simulink model "MMC_30_VSG_AD"  (R2023b)
settings: Solver=ode23t  StartTime=0.0  StopTime=2.4  RelTol=1e-3
InitFcn:
  | Rf=0.5929;
  | fn=50;
  | w0=2*pi*fn;
  | Lf=0.5*0.0135+0.01358;
  | R=0.5;
  | kf=8.5;
  | 
  | Kd=1.40543e+07;
  | lam=10; z0=0.707; zmax=1; wn0=lam/z0;
  | J0=223.613; DS0=4472.27;
  | Jmin=0.3*J0; Jmax=2.0*J0; Dmin=0.3*DS0; Dmax=2.2*DS0;
  | muJ=2906.97;
  | nu=0.15; nb=0.55; dzr=0.5; dzd=0;
  | tau=0.02; db=0.02; kpsi=14; txi=0.04;
  | Ts=0.0002; qref=0.03; dfref=0.064; dwref=0.4; dref=4;
  | lam_floor=1; scheme=1;
  | delta0=0.0712129;
  | J=J0; D=DS0;
libraries: spsIGBTDiodeLib x264, spsSeriesRLCBranchLib x140, spsVoltageMeasurementLib x132, spsCurrentMeasurementLib x6, spsSecondOrderFilterLib x3, spsThreePhaseVIMeasurementLib x2, spsDCVoltageSourceLib x2, slpidlib x2, spsGroundLib x1, spsPower3phInstantaneousLib x1, spsThreePhaseProgrammableVoltageSourceLib x1, spsThreePhaseSeriesRLCBranchLib x1
(part 1 of 5)
settings Model: Creator=LENOVO  LastModifiedBy=Lenovo
settings DataIOCC: ReturnWorkspaceOutputs=off

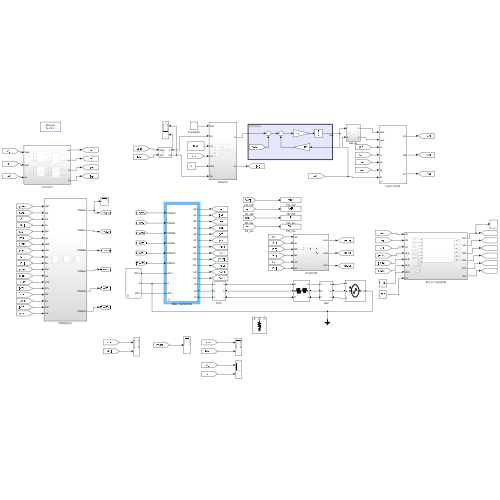
[thumbnail: Simulink's stored preview of the top-level diagram]
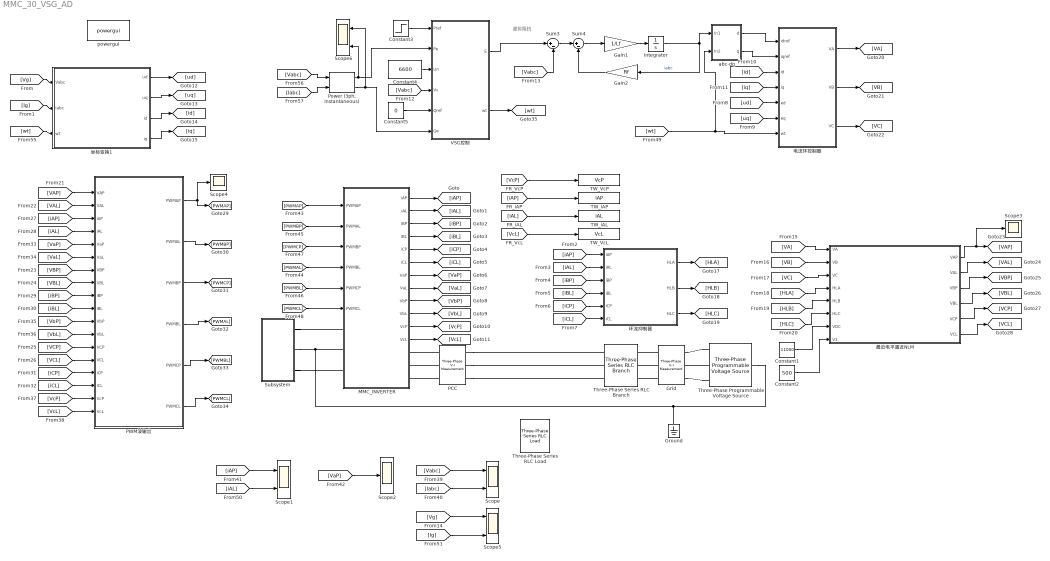
== system MMC_30_VSG_AD ==
  note: 虚拟阻抗
  Constant1 : Constant  Value=11000
  Constant2 : Constant  Value=500
  Constant3 : Step  Time=1.3  Before=1e6  After=1.1e6  SampleTime=0
  Constant4 : Constant  Value=6600
  Constant5 : Constant  Value=0
  Gain1 : Gain  Gain=1/Lf
  Gain2 : Gain  Gain=Rf
  Grid : spsThreePhaseVIMeasurementLib/Three-Phase V-I Measurement  VoltageMeasurement=phase-to-ground  SetLabelV=on  LabelV=Vg  Vpu=off  VpuLL=off  CurrentMeasurement=yes  SetLabelI=on  LabelI=Ig  Ipu=off  Pbase=100e6  Vbase=500e3  OutputType=Complex  PhasorSimulation=off  PSBequivalent=0
  Ground : spsGroundLib/Ground  LConnTagsString=a
  Integrator : Integrator
  MMC_INVERTER : Subsystem  mask{C0=4.7e-3, V0=500, L0=0.0135, C1=1e-3, R1=1e-6, V1=3500}
      mask prompts: C0 "旁路电容C0："; V0 "子模块初始电压V0："; L0 "桥臂电感L0："; C1 "直流电容C1："; R1 "电阻R1："; V1 "直流电容初始电压V1："
      mask DialogControl ParameterGroupVar Prompt: 参数
  PCC : spsThreePhaseVIMeasurementLib/Three-Phase V-I Measurement  VoltageMeasurement=phase-to-ground  SetLabelV=on  LabelV=Vabc  Vpu=off  VpuLL=off  CurrentMeasurement=yes  SetLabelI=on  LabelI=Iabc  Ipu=off  Pbase=100e6  Vbase=500e3  OutputType=Complex  PhasorSimulation=off  PSBequivalent=0
  PWM波输出 : Subsystem
  "Power (3ph, Instantaneous)" : spsPower3phInstantaneousLib/Power (3ph, Instantaneous)
  Scope{,1,5..6} (4 alike) : Scope  NumInputPorts=2
  Scope2 : Scope
  Scope3 : Scope
  Scope4 : Scope
  Subsystem : Subsystem  mask{VDC=11000}
      mask prompts: VDC "直流电压VDC："
      mask DialogControl ParameterGroupVar Prompt: 参数
  Sum3 : Sum  Inputs=|+-
  Sum4 : Sum  Inputs=|+-
  TW_VcL : ToWorkspace  VariableName=VcL  SaveFormat=Timeseries  SampleTime=Ts
  TW_VcP : ToWorkspace  VariableName=VcP  SaveFormat=Timeseries  SampleTime=Ts
  TW_iAL : ToWorkspace  VariableName=iAL  SaveFormat=Timeseries  SampleTime=Ts
  TW_iAP : ToWorkspace  VariableName=iAP  SaveFormat=Timeseries  SampleTime=Ts
  Three-Phase Programmable Voltage Source : spsThreePhaseProgrammableVoltageSourceLib/Three-Phase Programmable Voltage Source  PositiveSequence="[6600  0 50]"  VariationEntity=None  VariationType=Step  VariationTypeAlt=Step  VariationStep=-0.02  VariationRate=10  VariationMagnitude=0.3  VariationFrequency=2  VariationTiming=[1 2]  VariationPhaseA=off  Amplitudes=[1 0.8 1.2 1.0]  TimeValues=[0 0.1 0.15 0.2]  HarmonicGeneration=off  HarmonicA=[3 0.2 -25 0]  HarmonicB=[2 0.15 35 2]  Timing="[0.05  3]"  BusType=swing  Pref=0  Qref=0  Qmin=-inf  Qmax=inf
  Three-Phase Series RLC Branch : spsThreePhaseSeriesRLCBranchLib/Three-Phase Series RLC Branch  LConnTagsString=A|B|C  RConnTagsString=A|B|C  BranchType=RL  Resistance=0.5929  Inductance=13.58e-3  Capacitance=1e-6  Measurements=None
  Three-Phase Series RLC Load : spsThreePhaseSeriesRLCLoadLib/Three-Phase Series RLC Load  LConnTagsString=A|B|C  Configuration=Y (grounded)  NominalVoltage=6600  Vabc=[1e3 1e3 1e3]  Vabcp=[1e3 1e3 1e3]  NominalFrequency=50  UnbalancedPower=off  ActivePower=200e3  InductivePower=0  CapacitivePower=0  Pabc=[10e3 9e3 11e3]  QLabc=[100 90 110]  QCabc=[100 90 110]  Pabcp=[10e3 9e3 11e3]  QLabcp=[100 90 110]  QCabcp=[100 90 110]  Measurements=None  LoadType=constant Z
  VSG控制 : Subsystem
  abc-dq : Subsystem
  powergui : spspowerguiLib/powergui  Priority=1  SimulationMode=Discrete  SampleTime=5e-5  frequency=60  Iterations=50  frequencyindice=0  Pbase=100e6  ErrMax=1e-4  UnitsV=kV  UnitsW=MW  buscounter=0  FunctionMessages=off  echomessages=off  EnableUseOfTLC=off  CurrentSourceSwitches=off  DisableSnubberDevices=off  DisableRonSwitches=off  DisableVfSwitches=off  DisplayEquations=off  AutomaticDiscreteSolvers=off  SolverType=Tustin/Backward Euler (TBE)  Interpol=off  ExternalGateDelay=off  methode=off  Ts=100  x0status=blocks  SPID=on  SwTol=0  HookPort=off  NonlinearTolerance=1e-4  nMaxIteration=100  ContinueOnMaxIteration=off  RestoreLinks=warning  ResistiveCurrentMeasurement=off  Frange=[0:2:500]  Ylog=off  Xlog=on  ShowGrid=off  save=off  variable=ZData  structure=0  ZoomFFT=off  StartTime=0.0  cycles=1  DisplayStyle=1  fundamental=60  FreqAxis=off  MaxFrequency=1000  frequencyindicesteady=1  RmsSteady=1  display=off
  坐标变换1 : Subsystem
  最近电平逼近NLM : Subsystem
  环流抑制器 : Subsystem
  电流环控制器 : Subsystem  mask{Kp2=13.857, Ki2=58.576, wL=(0.0135/2+0.01358)*100*pi}
      mask prompts: Kp2 "电流内环Kp2："; Ki2 "电流内环Ki2："; wL "耦合量wL："
      mask DialogControl ParameterGroupVar Prompt: 参数
  wires:
  MMC_INVERTER/1(iAP) -> [iAP]
  MMC_INVERTER/2(iAL) -> [iAL]
  MMC_INVERTER/3(iBP) -> [iBP]
  MMC_INVERTER/4(iBL) -> [iBL]
  MMC_INVERTER/5(iCP) -> [iCP]
  MMC_INVERTER/6(iCL) -> [iCL]
  MMC_INVERTER/7(VaP) -> [VaP]
  MMC_INVERTER/12(VcL) -> [VcL]
  MMC_INVERTER/11(VcP) -> [VcP]
  MMC_INVERTER/10(VbL) -> [VbL]
  MMC_INVERTER/9(VbP) -> [VbP]
  MMC_INVERTER/8(VaL) -> [VaL]
  [Vg] -> 坐标变换1/1(Vabc)
  [Ig] -> 坐标变换1/2(Iabc)
  坐标变换1/1(ud) -> [ud]
  坐标变换1/2(uq) -> [uq]
  坐标变换1/3(id) -> [id]
  坐标变换1/4(iq) -> [iq]
  [iAP] -> 环流抑制器/1(iAP)
  [iAL] -> 环流抑制器/2(iAL)
  [iBP] -> 环流抑制器/3(iBP)
  [iBL] -> 环流抑制器/4(iBL)
  [iCP] -> 环流抑制器/5(iCP)
  [iCL] -> 环流抑制器/6(iCL)
  环流抑制器/1(HLA) -> [HLA]
  环流抑制器/2(HLB) -> [HLB]
  环流抑制器/3(HLC) -> [HLC]
  [id] -> 电流环控制器/3(id)
  [iq] -> 电流环控制器/4(iq)
  [ud] -> 电流环控制器/5(ed)
  [uq] -> 电流环控制器/6(eq)
  电流环控制器/1(VA) -> [VA]
  电流环控制器/2(VB) -> [VB]
  电流环控制器/3(VC) -> [VC]
  [VAP] -> PWM波输出/1(VAP)
  [VAL] -> PWM波输出/2(VAL)
  [VBP] -> PWM波输出/7(VBP)
  [VBL] -> PWM波输出/8(VBL)
  [VCP] -> PWM波输出/13(VCP)
  [VCL] -> PWM波输出/14(VCL)
  [iAP] -> PWM波输出/3(iAP)
  [iAL] -> PWM波输出/4(iAL)
  [VaP] -> PWM波输出/5(VaP)
  [VaL] -> PWM波输出/6(VaL)
  [iBP] -> PWM波输出/9(iBP)
  [iBL] -> PWM波输出/10(iBL)
  [VbP] -> PWM波输出/11(VbP)
  [VbL] -> PWM波输出/12(VbL)
  [iCP] -> PWM波输出/15(iCP)
  [iCL] -> PWM波输出/16(iCL)
  [VcP] -> PWM波输出/17(VcP)
  [VcL] -> PWM波输出/18(VcL)
  [Vabc] -> Scope/1
  [Iabc] -> Scope/2
  [iAP] -> Scope1/1
  [VaP] -> Scope2/1
  PWM波输出/6(PWMCL) -> [PWMCL]
  PWM波输出/4(PWMBL) -> [PWMAL]
  PWM波输出/5(PWMCP) -> [PWMBL]
  PWM波输出/1(PWMAP) -> [PWMAP], Scope4/1
  PWM波输出/3(PWMBP) -> [PWMCP]
  PWM波输出/2(PWMAL) -> [PWMBP]
  [PWMBP] -> MMC_INVERTER/2(PWMAL)
  [PWMCL] -> MMC_INVERTER/6(PWMCL)
  [PWMBL] -> MMC_INVERTER/5(PWMCP)
  [PWMAP] -> MMC_INVERTER/1(PWMAP)
  [PWMCP] -> MMC_INVERTER/3(PWMBP)
  [PWMAL] -> MMC_INVERTER/4(PWMBL)
  [iAL] -> Scope1/2
  "Power (3ph, Instantaneous)"/2 -> Scope6/1, VSG控制/6(Qe)
  Constant4/1 -> VSG控制/3(Un)
  "Power (3ph, Instantaneous)"/1 -> Scope6/2, VSG控制/2(Pe)
  [Vabc] -> VSG控制/4(Vs)
  Constant5/1 -> VSG控制/5(Qref)
  Constant3/1 -> VSG控制/1(Pref)
  [wt] -> 坐标变换1/3(wt)
  [Vabc] -> "Power (3ph, Instantaneous)"/1
  [Iabc] -> "Power (3ph, Instantaneous)"/2
  [VC] -> 最近电平逼近NLM/3(VC)
  Constant2/1 -> 最近电平逼近NLM/8(V1)
  Constant1/1 -> 最近电平逼近NLM/7(VDC)
  [HLB] -> 最近电平逼近NLM/5(HLB)
  最近电平逼近NLM/5(VCP) -> [VCP]
  最近电平逼近NLM/1(VAP) -> Scope3/1, [VAP]
  [VB] -> 最近电平逼近NLM/2(VB)
  最近电平逼近NLM/4(VBL) -> [VBL]
  [HLC] -> 最近电平逼近NLM/6(HLC)
  [VA] -> 最近电平逼近NLM/1(VA)
  最近电平逼近NLM/2(VAL) -> [VAL]
  最近电平逼近NLM/6(VCL) -> [VCL]
  [HLA] -> 最近电平逼近NLM/4(HLA)
  最近电平逼近NLM/3(VBP) -> [VBP]
  VSG控制/2(wt) -> [wt]
  [wt] -> abc-dq/2(In2), 电流环控制器/7(wt)
  Gain2/1 -> Sum4/2
  VSG控制/1(E) -> Sum3/1
  Sum4/1 -> Gain1/1
  Sum3/1 -> Sum4/1
  Gain1/1 -> Integrator/1
  [Vabc] -> Sum3/2
  Integrator/1 -> abc-dq/1(In1), Gain2/1  "iabc"
  abc-dq/1(d) -> 电流环控制器/1(idref)
  abc-dq/2(q) -> 电流环控制器/2(iqref)
  [Ig] -> Scope5/2
  [Vg] -> Scope5/1
  [VcP] -> TW_VcP/1
  [iAP] -> TW_iAP/1
  [iAL] -> TW_iAL/1
  [VcL] -> TW_VcL/1
  connections:
  PCC/LConn1 -- MMC_INVERTER/RConn1
  PCC/LConn2 -- MMC_INVERTER/RConn2
  PCC/LConn3 -- MMC_INVERTER/RConn3
  Subsystem/RConn2 -- Three-Phase Programmable Voltage Source/LConn1 -- Ground/LConn1 -- MMC_INVERTER/LConn2
  Subsystem/RConn3 -- MMC_INVERTER/LConn3
  Subsystem/RConn1 -- MMC_INVERTER/LConn1
  PCC/RConn1 -- Three-Phase Series RLC Branch/LConn1
  PCC/RConn2 -- Three-Phase Series RLC Branch/LConn2
  PCC/RConn3 -- Three-Phase Series RLC Branch/LConn3
  Grid/LConn1 -- Three-Phase Series RLC Branch/RConn1
  Grid/LConn2 -- Three-Phase Series RLC Branch/RConn2
  Grid/LConn3 -- Three-Phase Series RLC Branch/RConn3
  Three-Phase Programmable Voltage Source/RConn1 -- Grid/RConn1
  Three-Phase Programmable Voltage Source/RConn2 -- Grid/RConn2
  Three-Phase Programmable Voltage Source/RConn3 -- Grid/RConn3

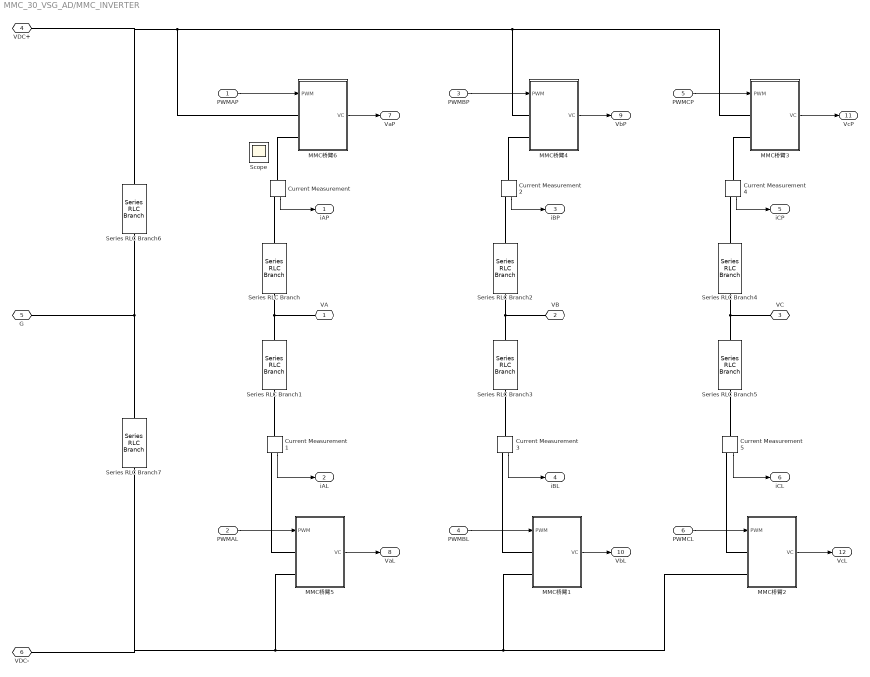
== system MMC_30_VSG_AD/MMC_INVERTER ==
  PWMAP : Inport
  PWMAL : Inport  Port=2
  PWMBP : Inport  Port=3
  PWMBL : Inport  Port=4
  PWMCP : Inport  Port=5
  PWMCL : Inport  Port=6
  Current Measurement{,1..5} (6 alike) : spsCurrentMeasurementLib/Current Measurement  PhasorSimulation=off  OutputType=Complex  PSBequivalent=0
  MMC桥臂1 : Subsystem
  MMC桥臂2 : Subsystem
  MMC桥臂3 : Subsystem
  MMC桥臂4 : Subsystem
  MMC桥臂5 : Subsystem
  MMC桥臂6 : Subsystem
  Scope : Scope
  Series RLC Branch{,1..5} (6 alike) : spsSeriesRLCBranchLib/Series RLC Branch  LConnTagsString=__new0  RConnTagsString=__new0  BranchType=L  Resistance=1  Inductance=L0  SetiL0=off  InitialCurrent=0  Capacitance=1e-6  Setx0=off  InitialVoltage=0  Measurements=None
  Series RLC Branch6 : spsSeriesRLCBranchLib/Series RLC Branch  LConnTagsString=__new0  RConnTagsString=__new0  BranchType=RC  Resistance=R1  Inductance=L0  SetiL0=off  InitialCurrent=0  Capacitance=2*C1  Setx0=on  InitialVoltage=V1/2  Measurements=None
  Series RLC Branch7 : spsSeriesRLCBranchLib/Series RLC Branch  LConnTagsString=__new0  RConnTagsString=__new0  BranchType=RC  Resistance=R1  Inductance=L0  SetiL0=off  InitialCurrent=0  Capacitance=2*C1  Setx0=on  InitialVoltage=V1/2  Measurements=None
  VA : PMIOPort  Side=Right
  VB : PMIOPort  Port=2  Side=Right
  VC : PMIOPort  Port=3  Side=Right
  VDC+ : PMIOPort  Port=4  Side=Left
  G : PMIOPort  Port=5  Side=Left
  VDC- : PMIOPort  Port=6  Side=Left
  iAP : Outport
  iAL : Outport  Port=2
  iBP : Outport  Port=3
  iBL : Outport  Port=4
  iCP : Outport  Port=5
  iCL : Outport  Port=6
  VaP : Outport  Port=7
  VaL : Outport  Port=8
  VbP : Outport  Port=9
  VbL : Outport  Port=10
  VcP : Outport  Port=11
  VcL : Outport  Port=12
  wires:
  MMC桥臂5/1(VC) -> VaL/1
  PWMAP/1 -> MMC桥臂6/1(PWM)
  MMC桥臂4/1(VC) -> VbP/1
  MMC桥臂6/1(VC) -> VaP/1
  MMC桥臂2/1(VC) -> VcL/1
  PWMCP/1 -> MMC桥臂3/1(PWM)
  PWMAL/1 -> MMC桥臂5/1(PWM)
  Current Measurement3/1 -> iBL/1
  MMC桥臂3/1(VC) -> VcP/1
  Current Measurement5/1 -> iCL/1
  PWMBL/1 -> MMC桥臂1/1(PWM)
  Current Measurement2/1 -> iBP/1
  PWMBP/1 -> MMC桥臂4/1(PWM)
  Current Measurement1/1 -> iAL/1
  Current Measurement/1 -> iAP/1
  PWMCL/1 -> MMC桥臂2/1(PWM)
  Current Measurement4/1 -> iCP/1
  MMC桥臂1/1(VC) -> VbL/1
  connections:
  MMC桥臂6/LConn2 -- Current Measurement/LConn1
  Series RLC Branch3/LConn1 -- VB/RConn1 -- Series RLC Branch2/RConn1
  Series RLC Branch/LConn1 -- Current Measurement/RConn1
  Current Measurement5/LConn1 -- Series RLC Branch5/RConn1
  VDC-/RConn1 -- Series RLC Branch7/RConn1 -- MMC桥臂5/LConn2 -- MMC桥臂2/LConn2 -- MMC桥臂1/LConn2
  Series RLC Branch1/LConn1 -- VA/RConn1 -- Series RLC Branch/RConn1
  Series RLC Branch5/LConn1 -- VC/RConn1 -- Series RLC Branch4/RConn1
  MMC桥臂5/LConn1 -- Current Measurement1/RConn1
  VDC+/RConn1 -- Series RLC Branch6/LConn1 -- MMC桥臂6/LConn1 -- MMC桥臂4/LConn1 -- MMC桥臂3/LConn1
  Series RLC Branch2/LConn1 -- Current Measurement2/RConn1
  MMC桥臂1/LConn1 -- Current Measurement3/RConn1
  MMC桥臂4/LConn2 -- Current Measurement2/LConn1
  Series RLC Branch4/LConn1 -- Current Measurement4/RConn1
  Current Measurement3/LConn1 -- Series RLC Branch3/RConn1
  Current Measurement1/LConn1 -- Series RLC Branch1/RConn1
  Series RLC Branch6/RConn1 -- G/RConn1 -- Series RLC Branch7/LConn1
  MMC桥臂2/LConn1 -- Current Measurement5/RConn1
  MMC桥臂3/LConn2 -- Current Measurement4/LConn1

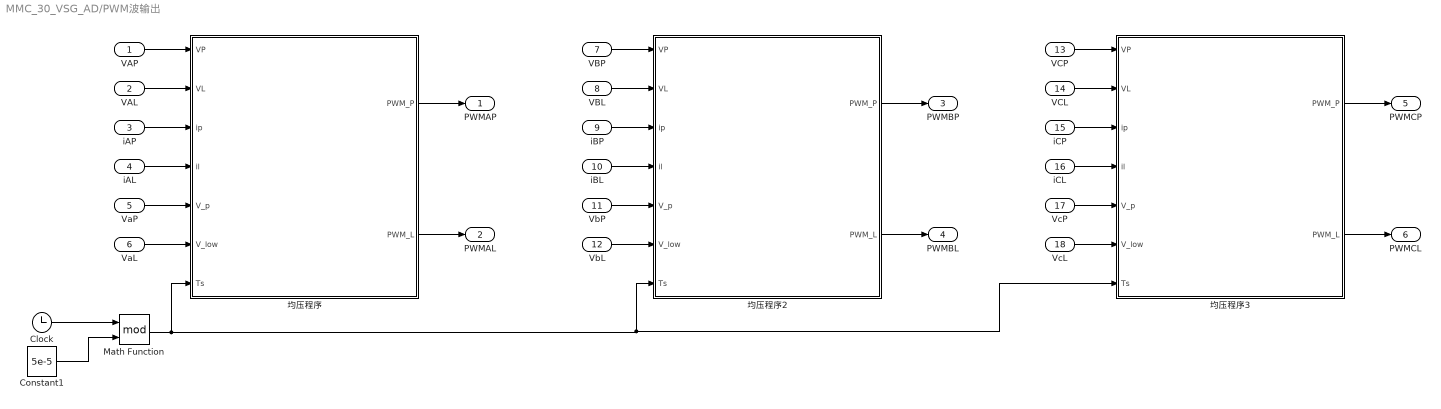
== system MMC_30_VSG_AD/PWM波输出 ==
  VAP : Inport
  VAL : Inport  Port=2
  iAP : Inport  Port=3
  iAL : Inport  Port=4
  VaP : Inport  Port=5
  VaL : Inport  Port=6
  VBP : Inport  Port=7
  VBL : Inport  Port=8
  iBP : Inport  Port=9
  iBL : Inport  Port=10
  VbP : Inport  Port=11
  VbL : Inport  Port=12
  VCP : Inport  Port=13
  VCL : Inport  Port=14
  iCP : Inport  Port=15
  iCL : Inport  Port=16
  VcP : Inport  Port=17
  VcL : Inport  Port=18
  Clock : Clock
  Constant1 : Constant  Value=5e-5
  Math Function : Math  Operator=mod
  均压程序 : MATLAB Function  TreatAsAtomicUnit=on
  均压程序2 : MATLAB Function  TreatAsAtomicUnit=on
  均压程序3 : MATLAB Function  TreatAsAtomicUnit=on
  PWMAP : Outport
  PWMAL : Outport  Port=2
  PWMBP : Outport  Port=3
  PWMBL : Outport  Port=4
  PWMCP : Outport  Port=5
  PWMCL : Outport  Port=6
  wires:
  VcL/1 -> 均压程序3/6(V_low)
  VAL/1 -> 均压程序/2(VL)
  均压程序3/2(PWM_L) -> PWMCL/1
  iBL/1 -> 均压程序2/4(il)
  Clock/1 -> Math Function/1
  均压程序3/1(PWM_P) -> PWMCP/1
  均压程序/1(PWM_P) -> PWMAP/1
  iCL/1 -> 均压程序3/4(il)
  iAP/1 -> 均压程序/3(ip)
  VcP/1 -> 均压程序3/5(V_p)
  VCL/1 -> 均压程序3/2(VL)
  VbP/1 -> 均压程序2/5(V_p)
  VAP/1 -> 均压程序/1(VP)
  VCP/1 -> 均压程序3/1(VP)
  iCP/1 -> 均压程序3/3(ip)
  VBP/1 -> 均压程序2/1(VP)
  Math Function/1 -> 均压程序3/7(Ts), 均压程序2/7(Ts), 均压程序/7(Ts)
  Constant1/1 -> Math Function/2
  均压程序2/1(PWM_P) -> PWMBP/1
  VaP/1 -> 均压程序/5(V_p)
  iAL/1 -> 均压程序/4(il)
  VBL/1 -> 均压程序2/2(VL)
  VaL/1 -> 均压程序/6(V_low)
  iBP/1 -> 均压程序2/3(ip)
  VbL/1 -> 均压程序2/6(V_low)
  均压程序/2(PWM_L) -> PWMAL/1
  均压程序2/2(PWM_L) -> PWMBL/1

== system MMC_30_VSG_AD/Subsystem ==
  DC Voltage Source : spsDCVoltageSourceLib/DC Voltage Source  Amplitude=VDC/2  Measurements=None
  DC Voltage Source1 : spsDCVoltageSourceLib/DC Voltage Source  Amplitude=VDC/2  Measurements=None
  VDC+ : PMIOPort  Side=Right
  G : PMIOPort  Port=2  Side=Right
  VDC- : PMIOPort  Port=3  Side=Right
  connections:
  DC Voltage Source1/RConn1 -- G/RConn1 -- DC Voltage Source/LConn1
  VDC-/RConn1 -- DC Voltage Source1/LConn1
  VDC+/RConn1 -- DC Voltage Source/RConn1

== system MMC_30_VSG_AD/VSG控制 ==
  note: 频率
  Pref : Inport
  Pe : Inport  Port=2
  Un : Inport  Port=3
  Vs : Inport  Port=4
  Qref : Inport  Port=5
  Qe : Inport  Port=6
  Constant : Constant  Value=[0 -2*pi/3 2*pi/3]
  Product : Product
  Scope : Scope
  Scope1 : Scope
  Sum : Sum  Inputs=|++
  Trigonometric Function : Trigonometry
  VSG无功控制-电压调节-调压 : Subsystem
  VSG有功控制-频率调节-一次调频 : Subsystem
  E : Outport
  wt : Outport  Port=2
  wires:
  Constant/1 -> Sum/2
  VSG有功控制-频率调节-一次调频/1(f) -> Scope/1
  Un/1 -> VSG无功控制-电压调节-调压/1(Un)
  Sum/1 -> Trigonometric Function/1
  Qe/1 -> VSG无功控制-电压调节-调压/4(Qe)
  Vs/1 -> VSG无功控制-电压调节-调压/2(Vs)
  Qref/1 -> VSG无功控制-电压调节-调压/3(Qref)
  Pref/1 -> VSG有功控制-频率调节-一次调频/1(Pref)
  Pe/1 -> VSG有功控制-频率调节-一次调频/2(Pe)
  Trigonometric Function/1 -> Product/1
  VSG无功控制-电压调节-调压/1(E) -> Product/2
  VSG有功控制-频率调节-一次调频/2(wt) -> wt/1, Sum/1
  Product/1 -> Scope1/1, E/1

== system MMC_30_VSG_AD/abc-dq ==
  In1 : Inport
  In2 : Inport  Port=2
  Demux : Demux  Outputs=3
  MATLAB Function : MATLAB Function  TreatAsAtomicUnit=on
  MATLAB Function1 : MATLAB Function  TreatAsAtomicUnit=on
  d : Outport
  q : Outport  Port=2
  wires:
  MATLAB Function/2(beta) -> MATLAB Function1/2(beta)
  MATLAB Function/1(alpha) -> MATLAB Function1/1(alpha)
  Demux/2 -> MATLAB Function/2(b)
  Demux/3 -> MATLAB Function/3(c)
  MATLAB Function1/2(q) -> q/1
  In2/1 -> MATLAB Function1/3(wt)
  Demux/1 -> MATLAB Function/1(a)
  MATLAB Function1/1(d) -> d/1
  In1/1 -> Demux/1

== system MMC_30_VSG_AD/坐标变换1 ==
  Vabc : Inport
  Iabc : Inport  Port=2
  wt : Inport  Port=3
  Demux : Demux  Outputs=3
  Demux1 : Demux  Outputs=3
  abctoalpha/beta : MATLAB Function  TreatAsAtomicUnit=on
  abctoalpha/beta1 : MATLAB Function  TreatAsAtomicUnit=on
  dq : MATLAB Function  TreatAsAtomicUnit=on
  dq1 : MATLAB Function  TreatAsAtomicUnit=on
  ud : Outport
  uq : Outport  Port=2
  id : Outport  Port=3
  iq : Outport  Port=4
  wires:
  abctoalpha/beta/1(alpha) -> dq/1(alpha)
  abctoalpha/beta1/2(beta) -> dq1/2(beta)
  dq1/1(d) -> id/1
  Demux/3 -> abctoalpha/beta/3(c)
  Vabc/1 -> Demux/1
  dq1/2(q) -> iq/1
  Demux/2 -> abctoalpha/beta/2(b)
  Demux1/2 -> abctoalpha/beta1/2(b)
  abctoalpha/beta/2(beta) -> dq/2(beta)
  wt/1 -> dq1/3(wt), dq/3(wt)
  Demux1/3 -> abctoalpha/beta1/3(c)
  Demux1/1 -> abctoalpha/beta1/1(a)
  Demux/1 -> abctoalpha/beta/1(a)
  abctoalpha/beta1/1(alpha) -> dq1/1(alpha)
  dq/2(q) -> uq/1
  Iabc/1 -> Demux1/1
  dq/1(d) -> ud/1

== system MMC_30_VSG_AD/最近电平逼近NLM ==
  VA : Inport
  VB : Inport  Port=2
  VC : Inport  Port=3
  HLA : Inport  Port=4
  HLB : Inport  Port=5
  HLC : Inport  Port=6
  VDC : Inport  Port=7
  V1 : Inport  Port=8
  NLM : MATLAB Function  TreatAsAtomicUnit=on
  VAP : Outport
  VAL : Outport  Port=2
  VBP : Outport  Port=3
  VBL : Outport  Port=4
  VCP : Outport  Port=5
  VCL : Outport  Port=6
  wires:
  NLM/2(VAL) -> VAL/1
  VC/1 -> NLM/3(VC)
  NLM/4(VBL) -> VBL/1
  HLA/1 -> NLM/4(HLA)
  VB/1 -> NLM/2(VB)
  NLM/1(VAP) -> VAP/1
  VA/1 -> NLM/1(VA)
  HLB/1 -> NLM/5(HLB)
  NLM/3(VBP) -> VBP/1
  HLC/1 -> NLM/6(HLC)
  NLM/5(VCP) -> VCP/1
  NLM/6(VCL) -> VCL/1
  VDC/1 -> NLM/7(VDC)
  V1/1 -> NLM/8(V1)

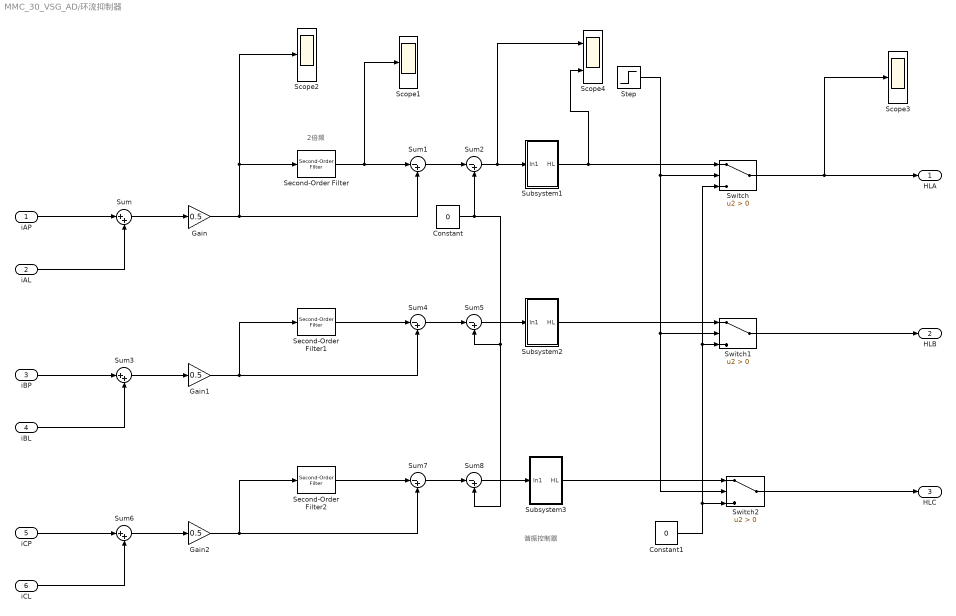
== system MMC_30_VSG_AD/环流抑制器 ==
  note: 2倍频
  note: 谐振控制器
  iAP : Inport
  iAL : Inport  Port=2
  iBP : Inport  Port=3
  iBL : Inport  Port=4
  iCP : Inport  Port=5
  iCL : Inport  Port=6
  Constant : Constant  Value=0
  Constant1 : Constant  Value=0
  Gain : Gain  Gain=0.5
  Gain1 : Gain  Gain=0.5
  Gain2 : Gain  Gain=0.5
  Scope1 : Scope
  Scope2 : Scope
  Scope3 : Scope
  Scope4 : Scope  NumInputPorts=2
  Second-Order Filter : spsSecondOrderFilterLib/Second-Order Filter  FilterType=Lowpass  Fo=10  Zeta=0.707  Ts=0  Initialize=off  Vac_Init="[0,  0,  60]"  Vdc_Init=0  PlotResponse=off  FreqRange=[0, 500, 1]
      settings: LibrarySourceBlock=|
      | sps_lib/Control/Filters/Second-Order
      | Filter
  Second-Order Filter1 : spsSecondOrderFilterLib/Second-Order Filter  FilterType=Lowpass  Fo=10  Zeta=0.707  Ts=0  Initialize=off  Vac_Init="[0,  0,  60]"  Vdc_Init=0  PlotResponse=off  FreqRange=[0, 500, 1]
      settings: LibrarySourceBlock=|
      | sps_lib/Control/Filters/Second-Order
      | Filter
  Second-Order Filter2 : spsSecondOrderFilterLib/Second-Order Filter  FilterType=Lowpass  Fo=10  Zeta=0.707  Ts=0  Initialize=off  Vac_Init="[0,  0,  60]"  Vdc_Init=0  PlotResponse=off  FreqRange=[0, 500, 1]
      settings: LibrarySourceBlock=|
      | sps_lib/Control/Filters/Second-Order
      | Filter
  Step : Step  Time=0.5  SampleTime=0
  Subsystem1 : Subsystem  mask{Kr=415, wr=2*50*2*pi, wc=5, Kp=120, Ki=0.1}
      mask prompts: Kr "谐振增益Kr："; wr "谐振频率wr："; wc "截至频率wc："; Kp "比例系数Kp："; Ki "积分系数Ki："
      mask DialogControl ParameterGroupVar Prompt: 参数
      mask Display: disp('PIR');
  Subsystem2 : Subsystem  mask{Kr=405, wr=2*50*2*pi, wc=5, Kp=120, Ki=0.1}
      mask prompts: Kr "谐振增益Kr："; wr "谐振频率wr："; wc "截至频率wc："; Kp "比例系数Kp："; Ki "积分系数Ki："
      mask DialogControl ParameterGroupVar Prompt: 参数
      mask Display: disp('PIR');
  Subsystem3 : Subsystem  mask{Kr=405, wr=2*50*2*pi, wc=5, Kp=120, Ki=0.1}
      mask prompts: Kr "谐振增益Kr："; wr "谐振频率wr："; wc "截至频率wc："; Kp "比例系数Kp："; Ki "积分系数Ki："
      mask DialogControl ParameterGroupVar Prompt: 参数
      mask Display: disp('PIR');
  Sum : Sum  Inputs=|++
  Sum{1..2,4..5,7..8} (6 alike) : Sum  Inputs=|-+
  Sum3 : Sum  Inputs=|++
  Sum6 : Sum  Inputs=|++
  Switch : Switch  Criteria=u2 > Threshold  SaturateOnIntegerOverflow=off  InputSameDT=off
  Switch1 : Switch  Criteria=u2 > Threshold  SaturateOnIntegerOverflow=off  InputSameDT=off
  Switch2 : Switch  Criteria=u2 > Threshold  SaturateOnIntegerOverflow=off  InputSameDT=off
  HLA : Outport
  HLB : Outport  Port=2
  HLC : Outport  Port=3
  wires:
  iBL/1 -> Sum3/2
  Sum/1 -> Gain/1
  Sum4/1 -> Sum5/1
  Sum2/1 -> Scope4/1, Subsystem1/1(In1)
  Constant/1 -> Sum8/2, Sum5/2, Sum2/2
  Sum5/1 -> Subsystem2/1(In1)
  Sum8/1 -> Subsystem3/1(In1)
  Sum1/1 -> Sum2/1
  iCL/1 -> Sum6/2
  iBP/1 -> Sum3/1
  Second-Order Filter/1 -> Scope1/1, Sum1/1
  Sum7/1 -> Sum8/1
  iAP/1 -> Sum/1
  Second-Order Filter1/1 -> Sum4/1
  iCP/1 -> Sum6/1
  Sum6/1 -> Gain2/1
  Second-Order Filter2/1 -> Sum7/1
  iAL/1 -> Sum/2
  Sum3/1 -> Gain1/1
  Switch/1 -> Scope3/1, HLA/1
  Subsystem3/1(HL) -> Switch2/1
  Subsystem2/1(HL) -> Switch1/1
  Subsystem1/1(HL) -> Scope4/2, Switch/1
  Switch1/1 -> HLB/1
  Switch2/1 -> HLC/1
  Constant1/1 -> Switch/3, Switch1/3, Switch2/3
  Step/1 -> Switch2/2, Switch1/2, Switch/2
  Gain2/1 -> Second-Order Filter2/1, Sum7/2
  Gain/1 -> Sum1/2, Scope2/1, Second-Order Filter/1
  Gain1/1 -> Second-Order Filter1/1, Sum4/2

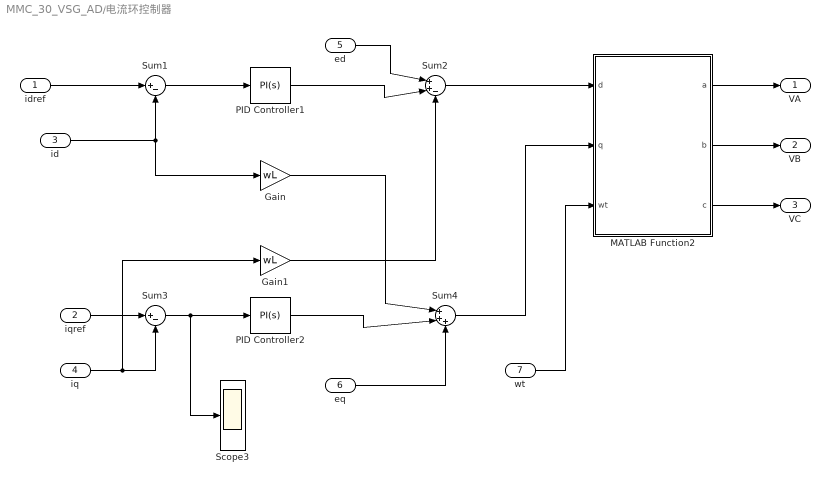
== system MMC_30_VSG_AD/电流环控制器 ==
  idref : Inport
  iqref : Inport  Port=2
  id : Inport  Port=3
  iq : Inport  Port=4
  ed : Inport  Port=5
  eq : Inport  Port=6
  wt : Inport  Port=7
  Gain : Gain  Gain=wL
  Gain1 : Gain  Gain=wL
  MATLAB Function2 : MATLAB Function  TreatAsAtomicUnit=on
  PID Controller1 : slpidlib/PID Controller  Controller=PI  Form=Parallel  TimeDomain=Continuous-time  UseExternalTs=off  SampleTime=-1  IntegratorMethod=Forward Euler  FilterMethod=Forward Euler  ControllerParametersSource=internal  P=Kp2  I=Ki2  UseKiTs=off  D=0  N=100  UseFilter=on  TunerSelectOption=Transfer Function Based (PID Tuner App)  InitialConditionSource=internal  InitialConditionForIntegrator=0  InitialConditionForFilter=0  DifferentiatorICPrevScaledInput=0  ExternalReset=none  TrackingMode=off  Kt=1  LimitOutput=off  SatLimitsSource=internal  UpperSaturationLimit=inf  LowerSaturationLimit=-inf  LinearizeAsGain=on  AntiWindupMode=none  Kb=1  LimitIntegrator=off  UpperIntegratorSaturationLimit=inf  LowerIntegratorSaturationLimit=-inf  POutMin=[]  POutMax=[]  IOutMin=[]  IOutMax=[]  DOutMin=[]  DOutMax=[]  NOutMin=[]  NOutMax=[]  SumOutMin=[]  SumOutMax=[]  SaturationOutMin=[]  SaturationOutMax=[]  PParamMin=[]  PParamMax=[]  IParamMin=[]  IParamMax=[]  DParamMin=[]  DParamMax=[]  NParamMin=[]  NParamMax=[]  KbParamMin=[]  KbParamMax=[]  KtParamMin=[]  KtParamMax=[]  KbOutMin=[]  KbOutMax=[]  KtOutMin=[]  KtOutMax=[]  IntegratorOutMin=[]  IntegratorOutMax=[]  FilterOutMin=[]  FilterOutMax=[]  SumI1OutMin=[]  SumI1OutMax=[]  SumI2OutMin=[]  SumI2OutMax=[]  SumI3OutMin=[]  SumI3OutMax=[]  SumI4OutMin=[]  SumI4OutMax=[]  SumDOutMin=[]  SumDOutMax=[]  DifferentiatorOutMin=[]  DifferentiatorOutMax=[]  FilterDiffOutCoefMin=[]  FilterDiffOutCoefMax=[]  ReciprocalOutMin=[]  ReciprocalOutMax=[]  SumDenOutMin=[]  SumDenOutMax=[]  SumNumOutMin=[]  SumNumOutMax=[]  DivideOutMin=[]  DivideOutMax=[]  UdiffTsProdOutMin=[]  UdiffTsProdOutMax=[]  NTsProdOutMin=[]  NTsProdOutMax=[]  UintegralTsProdOutMin=[]  UintegralTsProdOutMax=[]  UngainTsProdOutMin=[]  UngainTsProdOutMax=[]  ClampingZeroOutDataTypeStr=Inherit: Inherit via back propagation  ClampingZeroOutMin=[]  ClampingZeroOutMax=[]  FilterDenConstantOutDataTypeStr=Inherit: Inherit via back propagation  FilterDenConstantOutMin=[]  FilterDenConstantOutMax=[]  PCopyOutDataTypeStr=Inherit: Inherit via back propagation  PCopyOutMin=[]  PCopyOutMax=[]  NCopyOutDataTypeStr=Inherit: Inherit via back propagation  NCopyOutMin=[]  NCopyOutMax=[]  IntegratorContinuousStateAttributes=''  IntegratorStateMustResolveToSignalObject=off  IntegratorRTWStateStorageClass=Auto  FilterContinuousStateAttributes=''  FilterStateMustResolveToSignalObject=off  FilterRTWStateStorageClass=Auto  ParallelPVariant=InternalParameters  IdealPVariant=Disabled  IVariant=InternalParameters  DVariant=Disabled  IntegratorVariant=Continuous  SatVariant=Disabled  AWVariant=Passthrough  PCopyVariant=Disabled  TRVariant=Disabled  FdbkBlocksVariant=Forward  IdealPFdbkVariant=Disabled  SatFdbkVariant=Disabled  DerivativeFilterVariant=Disabled  NVariant=Disabled  NCopyVariant=Disabled_SignalSpec  FilterICVariant=Disabled  IntegratorICVariant=InternalICs  ExternalResetVariant=Disabled  TRSumVariant=Passthrough  SumFdbkVariant=Disabled  SumVariant=Sum_PI  TsampFilterVariant=InternalTs  TsampNgainVariant=Passthrough  TsampIntegralVariant=Disabled_SignalSpec  ExternalSaturationOutDataTypeStr=Inherit: Same as second input
  PID Controller2 : slpidlib/PID Controller  Controller=PI  Form=Parallel  TimeDomain=Continuous-time  UseExternalTs=off  SampleTime=-1  IntegratorMethod=Forward Euler  FilterMethod=Forward Euler  ControllerParametersSource=internal  P=Kp2  I=Ki2  UseKiTs=off  D=0  N=100  UseFilter=on  TunerSelectOption=Transfer Function Based (PID Tuner App)  InitialConditionSource=internal  InitialConditionForIntegrator=0  InitialConditionForFilter=0  DifferentiatorICPrevScaledInput=0  ExternalReset=none  TrackingMode=off  Kt=1  LimitOutput=off  SatLimitsSource=internal  UpperSaturationLimit=inf  LowerSaturationLimit=-inf  LinearizeAsGain=on  AntiWindupMode=none  Kb=1  LimitIntegrator=off  UpperIntegratorSaturationLimit=inf  LowerIntegratorSaturationLimit=-inf  POutMin=[]  POutMax=[]  IOutMin=[]  IOutMax=[]  DOutMin=[]  DOutMax=[]  NOutMin=[]  NOutMax=[]  SumOutMin=[]  SumOutMax=[]  SaturationOutMin=[]  SaturationOutMax=[]  PParamMin=[]  PParamMax=[]  IParamMin=[]  IParamMax=[]  DParamMin=[]  DParamMax=[]  NParamMin=[]  NParamMax=[]  KbParamMin=[]  KbParamMax=[]  KtParamMin=[]  KtParamMax=[]  KbOutMin=[]  KbOutMax=[]  KtOutMin=[]  KtOutMax=[]  IntegratorOutMin=[]  IntegratorOutMax=[]  FilterOutMin=[]  FilterOutMax=[]  SumI1OutMin=[]  SumI1OutMax=[]  SumI2OutMin=[]  SumI2OutMax=[]  SumI3OutMin=[]  SumI3OutMax=[]  SumI4OutMin=[]  SumI4OutMax=[]  SumDOutMin=[]  SumDOutMax=[]  DifferentiatorOutMin=[]  DifferentiatorOutMax=[]  FilterDiffOutCoefMin=[]  FilterDiffOutCoefMax=[]  ReciprocalOutMin=[]  ReciprocalOutMax=[]  SumDenOutMin=[]  SumDenOutMax=[]  SumNumOutMin=[]  SumNumOutMax=[]  DivideOutMin=[]  DivideOutMax=[]  UdiffTsProdOutMin=[]  UdiffTsProdOutMax=[]  NTsProdOutMin=[]  NTsProdOutMax=[]  UintegralTsProdOutMin=[]  UintegralTsProdOutMax=[]  UngainTsProdOutMin=[]  UngainTsProdOutMax=[]  ClampingZeroOutDataTypeStr=Inherit: Inherit via back propagation  ClampingZeroOutMin=[]  ClampingZeroOutMax=[]  FilterDenConstantOutDataTypeStr=Inherit: Inherit via back propagation  FilterDenConstantOutMin=[]  FilterDenConstantOutMax=[]  PCopyOutDataTypeStr=Inherit: Inherit via back propagation  PCopyOutMin=[]  PCopyOutMax=[]  NCopyOutDataTypeStr=Inherit: Inherit via back propagation  NCopyOutMin=[]  NCopyOutMax=[]  IntegratorContinuousStateAttributes=''  IntegratorStateMustResolveToSignalObject=off  IntegratorRTWStateStorageClass=Auto  FilterContinuousStateAttributes=''  FilterStateMustResolveToSignalObject=off  FilterRTWStateStorageClass=Auto  ParallelPVariant=InternalParameters  IdealPVariant=Disabled  IVariant=InternalParameters  DVariant=Disabled  IntegratorVariant=Continuous  SatVariant=Disabled  AWVariant=Passthrough  PCopyVariant=Disabled  TRVariant=Disabled  FdbkBlocksVariant=Forward  IdealPFdbkVariant=Disabled  SatFdbkVariant=Disabled  DerivativeFilterVariant=Disabled  NVariant=Disabled  NCopyVariant=Disabled_SignalSpec  FilterICVariant=Disabled  IntegratorICVariant=InternalICs  ExternalResetVariant=Disabled  TRSumVariant=Passthrough  SumFdbkVariant=Disabled  SumVariant=Sum_PI  TsampFilterVariant=InternalTs  TsampNgainVariant=Passthrough  TsampIntegralVariant=Disabled_SignalSpec  ExternalSaturationOutDataTypeStr=Inherit: Same as second input
  Scope3 : Scope
  Sum1 : Sum  Inputs=|+-
  Sum2 : Sum  Inputs=|++-
  Sum3 : Sum  Inputs=|+-
  Sum4 : Sum  Inputs=|+++
  VA : Outport
  VB : Outport  Port=2
  VC : Outport  Port=3
  wires:
  eq/1 -> Sum4/3
  Sum4/1 -> MATLAB Function2/2(q)
  PID Controller2/1 -> Sum4/2
  id/1 -> Gain/1, Sum1/2
  MATLAB Function2/3(c) -> VC/1
  Gain1/1 -> Sum2/3
  MATLAB Function2/1(a) -> VA/1
  MATLAB Function2/2(b) -> VB/1
  PID Controller1/1 -> Sum2/2
  Sum1/1 -> PID Controller1/1
  idref/1 -> Sum1/1
  iqref/1 -> Sum3/1
  iq/1 -> Gain1/1, Sum3/2
  Gain/1 -> Sum4/1
  wt/1 -> MATLAB Function2/3(wt)
  ed/1 -> Sum2/1
  Sum2/1 -> MATLAB Function2/1(d)
  Sum3/1 -> Scope3/1, PID Controller2/1

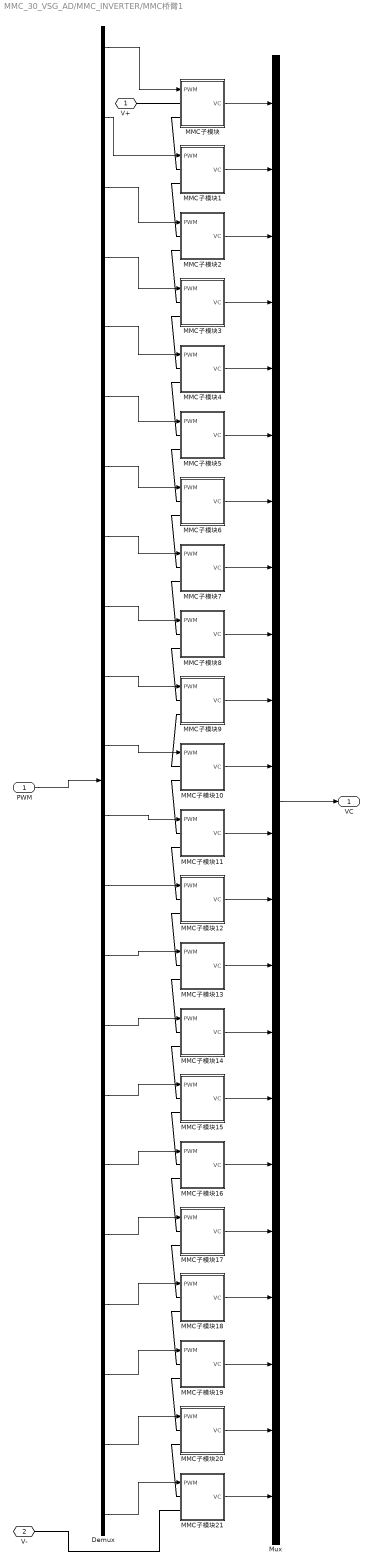
== system MMC_30_VSG_AD/MMC_INVERTER/MMC桥臂1 ==
  PWM : Inport
  Demux : Demux  Outputs=22
  MMC子模块 : Subsystem
  MMC子模块1 : Subsystem
  MMC子模块10 : Subsystem
  MMC子模块11 : Subsystem
  MMC子模块12 : Subsystem
  MMC子模块13 : Subsystem
  MMC子模块14 : Subsystem
  MMC子模块15 : Subsystem
  MMC子模块16 : Subsystem
  MMC子模块17 : Subsystem
  MMC子模块18 : Subsystem
  MMC子模块19 : Subsystem
  MMC子模块2 : Subsystem
  MMC子模块20 : Subsystem
  MMC子模块21 : Subsystem
  MMC子模块3 : Subsystem
  MMC子模块4 : Subsystem
  MMC子模块5 : Subsystem
  MMC子模块6 : Subsystem
  MMC子模块7 : Subsystem
  MMC子模块8 : Subsystem
  MMC子模块9 : Subsystem
  Mux : Mux  Inputs=22
  V+ : PMIOPort  Side=Left
  V- : PMIOPort  Port=2  Side=Left
  VC : Outport
  wires:
  MMC子模块20/1(VC) -> Mux/21
  MMC子模块18/1(VC) -> Mux/19
  Demux/14 -> MMC子模块13/1(PWM)
  Demux/5 -> MMC子模块4/1(PWM)
  MMC子模块6/1(VC) -> Mux/7
  PWM/1 -> Demux/1
  MMC子模块3/1(VC) -> Mux/4
  MMC子模块8/1(VC) -> Mux/9
  MMC子模块10/1(VC) -> Mux/11
  Demux/7 -> MMC子模块6/1(PWM)
  Demux/8 -> MMC子模块7/1(PWM)
  Demux/6 -> MMC子模块5/1(PWM)
  Demux/12 -> MMC子模块11/1(PWM)
  MMC子模块12/1(VC) -> Mux/13
  MMC子模块/1(VC) -> Mux/1
  Demux/18 -> MMC子模块17/1(PWM)
  MMC子模块15/1(VC) -> Mux/16
  Demux/15 -> MMC子模块14/1(PWM)
  MMC子模块13/1(VC) -> Mux/14
  MMC子模块21/1(VC) -> Mux/22
  Demux/11 -> MMC子模块10/1(PWM)
  Demux/9 -> MMC子模块8/1(PWM)
  Demux/10 -> MMC子模块9/1(PWM)
  Demux/4 -> MMC子模块3/1(PWM)
  MMC子模块5/1(VC) -> Mux/6
  MMC子模块11/1(VC) -> Mux/12
  Demux/3 -> MMC子模块2/1(PWM)
  MMC子模块2/1(VC) -> Mux/3
  MMC子模块17/1(VC) -> Mux/18
  MMC子模块19/1(VC) -> Mux/20
  MMC子模块16/1(VC) -> Mux/17
  Demux/20 -> MMC子模块19/1(PWM)
  MMC子模块1/1(VC) -> Mux/2
  Demux/2 -> MMC子模块1/1(PWM)
  Demux/13 -> MMC子模块12/1(PWM)
  MMC子模块7/1(VC) -> Mux/8
  Demux/16 -> MMC子模块15/1(PWM)
  MMC子模块9/1(VC) -> Mux/10
  Mux/1 -> VC/1
  MMC子模块14/1(VC) -> Mux/15
  Demux/1 -> MMC子模块/1(PWM)
  Demux/17 -> MMC子模块16/1(PWM)
  Demux/22 -> MMC子模块21/1(PWM)
  Demux/19 -> MMC子模块18/1(PWM)
  Demux/21 -> MMC子模块20/1(PWM)
  MMC子模块4/1(VC) -> Mux/5
  connections:
  V-/RConn1 -- MMC子模块21/LConn2
  V+/RConn1 -- MMC子模块/LConn1
  MMC子模块16/LConn2 -- MMC子模块17/LConn1
  MMC子模块18/LConn2 -- MMC子模块19/LConn1
  MMC子模块/LConn2 -- MMC子模块1/LConn1
  MMC子模块8/LConn2 -- MMC子模块9/LConn1
  MMC子模块11/LConn2 -- MMC子模块12/LConn1
  MMC子模块17/LConn2 -- MMC子模块18/LConn1
  MMC子模块12/LConn2 -- MMC子模块13/LConn1
  MMC子模块4/LConn2 -- MMC子模块5/LConn1
  MMC子模块20/LConn2 -- MMC子模块21/LConn1
  MMC子模块15/LConn2 -- MMC子模块16/LConn1
  MMC子模块19/LConn2 -- MMC子模块20/LConn1
  MMC子模块14/LConn2 -- MMC子模块15/LConn1
  MMC子模块7/LConn2 -- MMC子模块8/LConn1
  MMC子模块1/LConn2 -- MMC子模块2/LConn1
  MMC子模块10/LConn2 -- MMC子模块11/LConn1
  MMC子模块3/LConn2 -- MMC子模块4/LConn1
  MMC子模块5/LConn2 -- MMC子模块6/LConn1
  MMC子模块13/LConn2 -- MMC子模块14/LConn1
  MMC子模块2/LConn2 -- MMC子模块3/LConn1
  MMC子模块10/LConn1 -- MMC子模块9/LConn2
  MMC子模块6/LConn2 -- MMC子模块7/LConn1

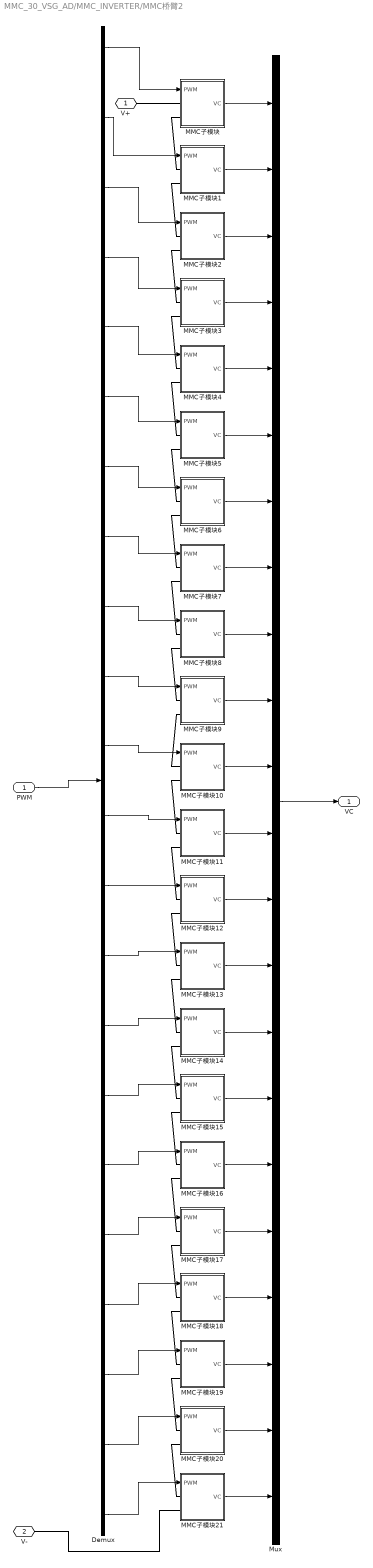
== system MMC_30_VSG_AD/MMC_INVERTER/MMC桥臂2 ==
  PWM : Inport
  Demux : Demux  Outputs=22
  MMC子模块 : Subsystem
  MMC子模块1 : Subsystem
  MMC子模块10 : Subsystem
  MMC子模块11 : Subsystem
  MMC子模块12 : Subsystem
  MMC子模块13 : Subsystem
  MMC子模块14 : Subsystem
  MMC子模块15 : Subsystem
  MMC子模块16 : Subsystem
  MMC子模块17 : Subsystem
  MMC子模块18 : Subsystem
  MMC子模块19 : Subsystem
  MMC子模块2 : Subsystem
  MMC子模块20 : Subsystem
  MMC子模块21 : Subsystem
  MMC子模块3 : Subsystem
  MMC子模块4 : Subsystem
  MMC子模块5 : Subsystem
  MMC子模块6 : Subsystem
  MMC子模块7 : Subsystem
  MMC子模块8 : Subsystem
  MMC子模块9 : Subsystem
  Mux : Mux  Inputs=22
  V+ : PMIOPort  Side=Left
  V- : PMIOPort  Port=2  Side=Left
  VC : Outport
  wires:
  MMC子模块4/1(VC) -> Mux/5
  Demux/21 -> MMC子模块20/1(PWM)
  Demux/19 -> MMC子模块18/1(PWM)
  Demux/22 -> MMC子模块21/1(PWM)
  Demux/17 -> MMC子模块16/1(PWM)
  Demux/1 -> MMC子模块/1(PWM)
  MMC子模块14/1(VC) -> Mux/15
  Mux/1 -> VC/1
  MMC子模块9/1(VC) -> Mux/10
  Demux/16 -> MMC子模块15/1(PWM)
  MMC子模块7/1(VC) -> Mux/8
  Demux/13 -> MMC子模块12/1(PWM)
  Demux/2 -> MMC子模块1/1(PWM)
  MMC子模块1/1(VC) -> Mux/2
  Demux/20 -> MMC子模块19/1(PWM)
  MMC子模块16/1(VC) -> Mux/17
  MMC子模块19/1(VC) -> Mux/20
  MMC子模块17/1(VC) -> Mux/18
  MMC子模块2/1(VC) -> Mux/3
  Demux/3 -> MMC子模块2/1(PWM)
  MMC子模块11/1(VC) -> Mux/12
  MMC子模块5/1(VC) -> Mux/6
  Demux/4 -> MMC子模块3/1(PWM)
  Demux/10 -> MMC子模块9/1(PWM)
  Demux/9 -> MMC子模块8/1(PWM)
  Demux/11 -> MMC子模块10/1(PWM)
  MMC子模块21/1(VC) -> Mux/22
  MMC子模块13/1(VC) -> Mux/14
  Demux/15 -> MMC子模块14/1(PWM)
  MMC子模块15/1(VC) -> Mux/16
  Demux/18 -> MMC子模块17/1(PWM)
  MMC子模块/1(VC) -> Mux/1
  MMC子模块12/1(VC) -> Mux/13
  Demux/12 -> MMC子模块11/1(PWM)
  Demux/6 -> MMC子模块5/1(PWM)
  Demux/8 -> MMC子模块7/1(PWM)
  Demux/7 -> MMC子模块6/1(PWM)
  MMC子模块10/1(VC) -> Mux/11
  MMC子模块8/1(VC) -> Mux/9
  MMC子模块3/1(VC) -> Mux/4
  PWM/1 -> Demux/1
  MMC子模块6/1(VC) -> Mux/7
  Demux/5 -> MMC子模块4/1(PWM)
  Demux/14 -> MMC子模块13/1(PWM)
  MMC子模块18/1(VC) -> Mux/19
  MMC子模块20/1(VC) -> Mux/21
  connections:
  MMC子模块6/LConn2 -- MMC子模块7/LConn1
  MMC子模块10/LConn1 -- MMC子模块9/LConn2
  MMC子模块2/LConn2 -- MMC子模块3/LConn1
  MMC子模块13/LConn2 -- MMC子模块14/LConn1
  MMC子模块5/LConn2 -- MMC子模块6/LConn1
  MMC子模块3/LConn2 -- MMC子模块4/LConn1
  MMC子模块10/LConn2 -- MMC子模块11/LConn1
  MMC子模块1/LConn2 -- MMC子模块2/LConn1
  MMC子模块7/LConn2 -- MMC子模块8/LConn1
  MMC子模块14/LConn2 -- MMC子模块15/LConn1
  MMC子模块19/LConn2 -- MMC子模块20/LConn1
  MMC子模块15/LConn2 -- MMC子模块16/LConn1
  MMC子模块20/LConn2 -- MMC子模块21/LConn1
  MMC子模块4/LConn2 -- MMC子模块5/LConn1
  MMC子模块12/LConn2 -- MMC子模块13/LConn1
  MMC子模块17/LConn2 -- MMC子模块18/LConn1
  MMC子模块11/LConn2 -- MMC子模块12/LConn1
  MMC子模块8/LConn2 -- MMC子模块9/LConn1
  MMC子模块/LConn2 -- MMC子模块1/LConn1
  MMC子模块18/LConn2 -- MMC子模块19/LConn1
  MMC子模块16/LConn2 -- MMC子模块17/LConn1
  V+/RConn1 -- MMC子模块/LConn1
  V-/RConn1 -- MMC子模块21/LConn2

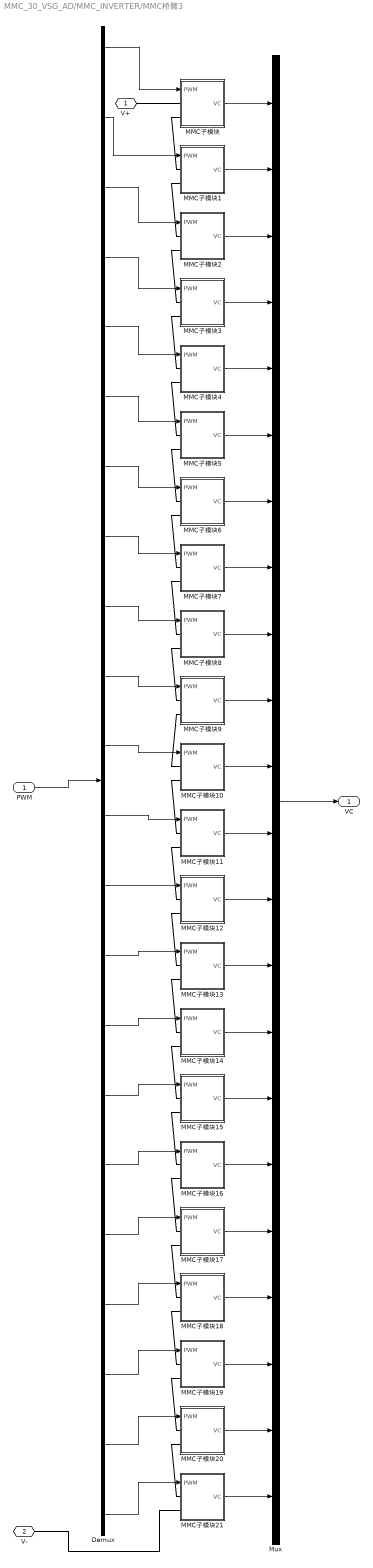
== system MMC_30_VSG_AD/MMC_INVERTER/MMC桥臂3 ==
  PWM : Inport
  Demux : Demux  Outputs=22
  MMC子模块 : Subsystem
  MMC子模块1 : Subsystem
  MMC子模块10 : Subsystem
  MMC子模块11 : Subsystem
  MMC子模块12 : Subsystem
  MMC子模块13 : Subsystem
  MMC子模块14 : Subsystem
  MMC子模块15 : Subsystem
  MMC子模块16 : Subsystem
  MMC子模块17 : Subsystem
  MMC子模块18 : Subsystem
  MMC子模块19 : Subsystem
  MMC子模块2 : Subsystem
  MMC子模块20 : Subsystem
  MMC子模块21 : Subsystem
  MMC子模块3 : Subsystem
  MMC子模块4 : Subsystem
  MMC子模块5 : Subsystem
  MMC子模块6 : Subsystem
  MMC子模块7 : Subsystem
  MMC子模块8 : Subsystem
  MMC子模块9 : Subsystem
  Mux : Mux  Inputs=22
  V+ : PMIOPort  Side=Left
  V- : PMIOPort  Port=2  Side=Left
  VC : Outport
  wires:
  MMC子模块20/1(VC) -> Mux/21
  MMC子模块18/1(VC) -> Mux/19
  Demux/14 -> MMC子模块13/1(PWM)
  Demux/5 -> MMC子模块4/1(PWM)
  MMC子模块6/1(VC) -> Mux/7
  PWM/1 -> Demux/1
  MMC子模块3/1(VC) -> Mux/4
  MMC子模块8/1(VC) -> Mux/9
  MMC子模块10/1(VC) -> Mux/11
  Demux/7 -> MMC子模块6/1(PWM)
  Demux/8 -> MMC子模块7/1(PWM)
  Demux/6 -> MMC子模块5/1(PWM)
  Demux/12 -> MMC子模块11/1(PWM)
  MMC子模块12/1(VC) -> Mux/13
  MMC子模块/1(VC) -> Mux/1
  Demux/18 -> MMC子模块17/1(PWM)
  MMC子模块15/1(VC) -> Mux/16
  Demux/15 -> MMC子模块14/1(PWM)
  MMC子模块13/1(VC) -> Mux/14
  MMC子模块21/1(VC) -> Mux/22
  Demux/11 -> MMC子模块10/1(PWM)
  Demux/9 -> MMC子模块8/1(PWM)
  Demux/10 -> MMC子模块9/1(PWM)
  Demux/4 -> MMC子模块3/1(PWM)
  MMC子模块5/1(VC) -> Mux/6
  MMC子模块11/1(VC) -> Mux/12
  Demux/3 -> MMC子模块2/1(PWM)
  MMC子模块2/1(VC) -> Mux/3
  MMC子模块17/1(VC) -> Mux/18
  MMC子模块19/1(VC) -> Mux/20
  MMC子模块16/1(VC) -> Mux/17
  Demux/20 -> MMC子模块19/1(PWM)
  MMC子模块1/1(VC) -> Mux/2
  Demux/2 -> MMC子模块1/1(PWM)
  Demux/13 -> MMC子模块12/1(PWM)
  MMC子模块7/1(VC) -> Mux/8
  Demux/16 -> MMC子模块15/1(PWM)
  MMC子模块9/1(VC) -> Mux/10
  Mux/1 -> VC/1
  MMC子模块14/1(VC) -> Mux/15
  Demux/1 -> MMC子模块/1(PWM)
  Demux/17 -> MMC子模块16/1(PWM)
  Demux/22 -> MMC子模块21/1(PWM)
  Demux/19 -> MMC子模块18/1(PWM)
  Demux/21 -> MMC子模块20/1(PWM)
  MMC子模块4/1(VC) -> Mux/5
  connections:
  V-/RConn1 -- MMC子模块21/LConn2
  V+/RConn1 -- MMC子模块/LConn1
  MMC子模块16/LConn2 -- MMC子模块17/LConn1
  MMC子模块18/LConn2 -- MMC子模块19/LConn1
  MMC子模块/LConn2 -- MMC子模块1/LConn1
  MMC子模块8/LConn2 -- MMC子模块9/LConn1
  MMC子模块11/LConn2 -- MMC子模块12/LConn1
  MMC子模块17/LConn2 -- MMC子模块18/LConn1
  MMC子模块12/LConn2 -- MMC子模块13/LConn1
  MMC子模块4/LConn2 -- MMC子模块5/LConn1
  MMC子模块20/LConn2 -- MMC子模块21/LConn1
  MMC子模块15/LConn2 -- MMC子模块16/LConn1
  MMC子模块19/LConn2 -- MMC子模块20/LConn1
  MMC子模块14/LConn2 -- MMC子模块15/LConn1
  MMC子模块7/LConn2 -- MMC子模块8/LConn1
  MMC子模块1/LConn2 -- MMC子模块2/LConn1
  MMC子模块10/LConn2 -- MMC子模块11/LConn1
  MMC子模块3/LConn2 -- MMC子模块4/LConn1
  MMC子模块5/LConn2 -- MMC子模块6/LConn1
  MMC子模块13/LConn2 -- MMC子模块14/LConn1
  MMC子模块2/LConn2 -- MMC子模块3/LConn1
  MMC子模块10/LConn1 -- MMC子模块9/LConn2
  MMC子模块6/LConn2 -- MMC子模块7/LConn1

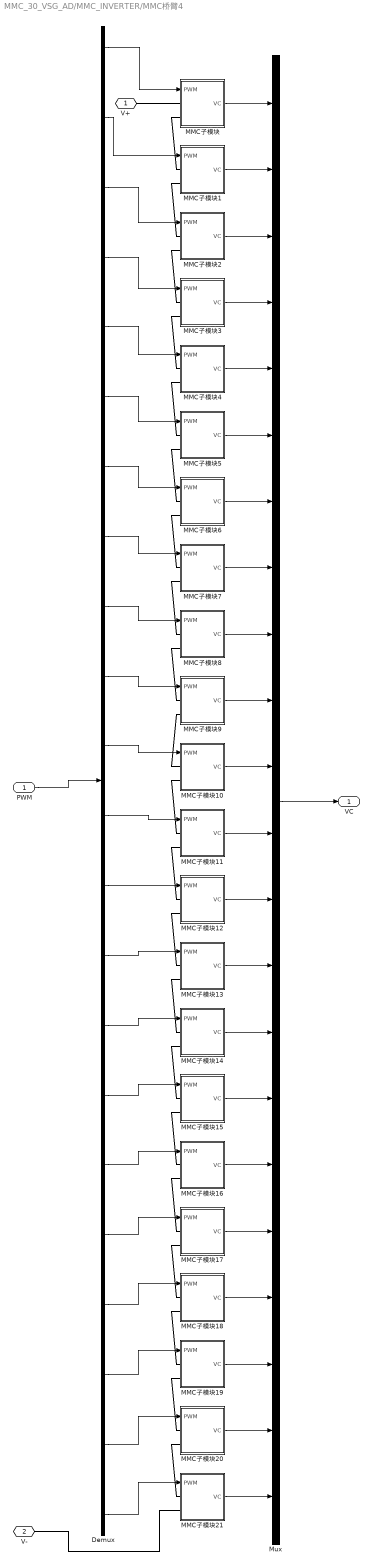
== system MMC_30_VSG_AD/MMC_INVERTER/MMC桥臂4 ==
  PWM : Inport
  Demux : Demux  Outputs=22
  MMC子模块 : Subsystem
  MMC子模块1 : Subsystem
  MMC子模块10 : Subsystem
  MMC子模块11 : Subsystem
  MMC子模块12 : Subsystem
  MMC子模块13 : Subsystem
  MMC子模块14 : Subsystem
  MMC子模块15 : Subsystem
  MMC子模块16 : Subsystem
  MMC子模块17 : Subsystem
  MMC子模块18 : Subsystem
  MMC子模块19 : Subsystem
  MMC子模块2 : Subsystem
  MMC子模块20 : Subsystem
  MMC子模块21 : Subsystem
  MMC子模块3 : Subsystem
  MMC子模块4 : Subsystem
  MMC子模块5 : Subsystem
  MMC子模块6 : Subsystem
  MMC子模块7 : Subsystem
  MMC子模块8 : Subsystem
  MMC子模块9 : Subsystem
  Mux : Mux  Inputs=22
  V+ : PMIOPort  Side=Left
  V- : PMIOPort  Port=2  Side=Left
  VC : Outport
  wires:
  MMC子模块4/1(VC) -> Mux/5
  Demux/21 -> MMC子模块20/1(PWM)
  Demux/19 -> MMC子模块18/1(PWM)
  Demux/22 -> MMC子模块21/1(PWM)
  Demux/17 -> MMC子模块16/1(PWM)
  Demux/1 -> MMC子模块/1(PWM)
  MMC子模块14/1(VC) -> Mux/15
  Mux/1 -> VC/1
  MMC子模块9/1(VC) -> Mux/10
  Demux/16 -> MMC子模块15/1(PWM)
  MMC子模块7/1(VC) -> Mux/8
  Demux/13 -> MMC子模块12/1(PWM)
  Demux/2 -> MMC子模块1/1(PWM)
  MMC子模块1/1(VC) -> Mux/2
  Demux/20 -> MMC子模块19/1(PWM)
  MMC子模块16/1(VC) -> Mux/17
  MMC子模块19/1(VC) -> Mux/20
  MMC子模块17/1(VC) -> Mux/18
  MMC子模块2/1(VC) -> Mux/3
  Demux/3 -> MMC子模块2/1(PWM)
  MMC子模块11/1(VC) -> Mux/12
  MMC子模块5/1(VC) -> Mux/6
  Demux/4 -> MMC子模块3/1(PWM)
  Demux/10 -> MMC子模块9/1(PWM)
  Demux/9 -> MMC子模块8/1(PWM)
  Demux/11 -> MMC子模块10/1(PWM)
  MMC子模块21/1(VC) -> Mux/22
  MMC子模块13/1(VC) -> Mux/14
  Demux/15 -> MMC子模块14/1(PWM)
  MMC子模块15/1(VC) -> Mux/16
  Demux/18 -> MMC子模块17/1(PWM)
  MMC子模块/1(VC) -> Mux/1
  MMC子模块12/1(VC) -> Mux/13
  Demux/12 -> MMC子模块11/1(PWM)
  Demux/6 -> MMC子模块5/1(PWM)
  Demux/8 -> MMC子模块7/1(PWM)
  Demux/7 -> MMC子模块6/1(PWM)
  MMC子模块10/1(VC) -> Mux/11
  MMC子模块8/1(VC) -> Mux/9
  MMC子模块3/1(VC) -> Mux/4
  PWM/1 -> Demux/1
  MMC子模块6/1(VC) -> Mux/7
  Demux/5 -> MMC子模块4/1(PWM)
  Demux/14 -> MMC子模块13/1(PWM)
  MMC子模块18/1(VC) -> Mux/19
  MMC子模块20/1(VC) -> Mux/21
  connections:
  MMC子模块6/LConn2 -- MMC子模块7/LConn1
  MMC子模块10/LConn1 -- MMC子模块9/LConn2
  MMC子模块2/LConn2 -- MMC子模块3/LConn1
  MMC子模块13/LConn2 -- MMC子模块14/LConn1
  MMC子模块5/LConn2 -- MMC子模块6/LConn1
  MMC子模块3/LConn2 -- MMC子模块4/LConn1
  MMC子模块10/LConn2 -- MMC子模块11/LConn1
  MMC子模块1/LConn2 -- MMC子模块2/LConn1
  MMC子模块7/LConn2 -- MMC子模块8/LConn1
  MMC子模块14/LConn2 -- MMC子模块15/LConn1
  MMC子模块19/LConn2 -- MMC子模块20/LConn1
  MMC子模块15/LConn2 -- MMC子模块16/LConn1
  MMC子模块20/LConn2 -- MMC子模块21/LConn1
  MMC子模块4/LConn2 -- MMC子模块5/LConn1
  MMC子模块12/LConn2 -- MMC子模块13/LConn1
  MMC子模块17/LConn2 -- MMC子模块18/LConn1
  MMC子模块11/LConn2 -- MMC子模块12/LConn1
  MMC子模块8/LConn2 -- MMC子模块9/LConn1
  MMC子模块/LConn2 -- MMC子模块1/LConn1
  MMC子模块18/LConn2 -- MMC子模块19/LConn1
  MMC子模块16/LConn2 -- MMC子模块17/LConn1
  V+/RConn1 -- MMC子模块/LConn1
  V-/RConn1 -- MMC子模块21/LConn2

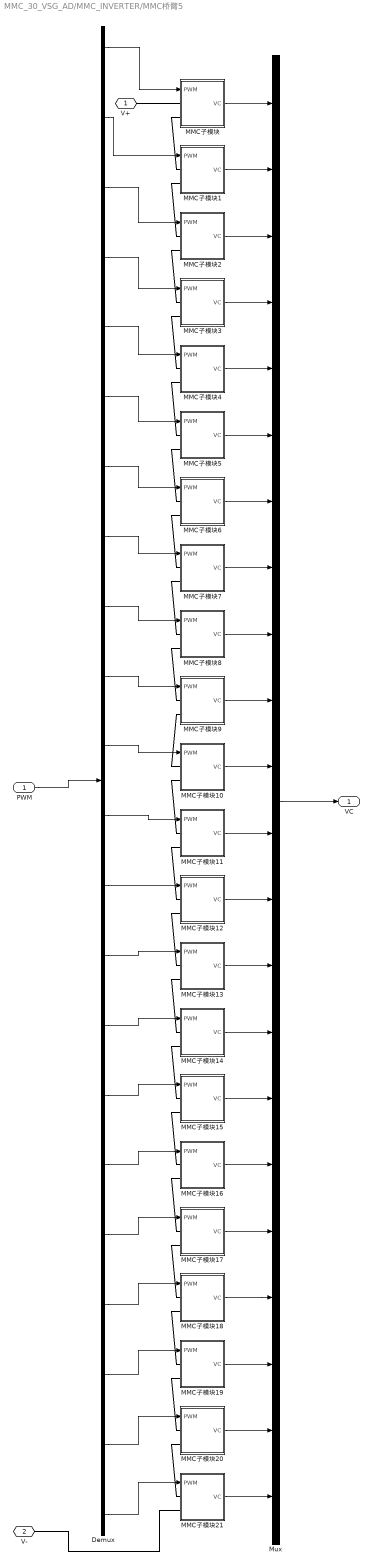
== system MMC_30_VSG_AD/MMC_INVERTER/MMC桥臂5 ==
  PWM : Inport
  Demux : Demux  Outputs=22
  MMC子模块 : Subsystem
  MMC子模块1 : Subsystem
  MMC子模块10 : Subsystem
  MMC子模块11 : Subsystem
  MMC子模块12 : Subsystem
  MMC子模块13 : Subsystem
  MMC子模块14 : Subsystem
  MMC子模块15 : Subsystem
  MMC子模块16 : Subsystem
  MMC子模块17 : Subsystem
  MMC子模块18 : Subsystem
  MMC子模块19 : Subsystem
  MMC子模块2 : Subsystem
  MMC子模块20 : Subsystem
  MMC子模块21 : Subsystem
  MMC子模块3 : Subsystem
  MMC子模块4 : Subsystem
  MMC子模块5 : Subsystem
  MMC子模块6 : Subsystem
  MMC子模块7 : Subsystem
  MMC子模块8 : Subsystem
  MMC子模块9 : Subsystem
  Mux : Mux  Inputs=22
  V+ : PMIOPort  Side=Left
  V- : PMIOPort  Port=2  Side=Left
  VC : Outport
  wires:
  MMC子模块4/1(VC) -> Mux/5
  Demux/21 -> MMC子模块20/1(PWM)
  Demux/19 -> MMC子模块18/1(PWM)
  Demux/22 -> MMC子模块21/1(PWM)
  Demux/17 -> MMC子模块16/1(PWM)
  Demux/1 -> MMC子模块/1(PWM)
  MMC子模块14/1(VC) -> Mux/15
  Mux/1 -> VC/1
  MMC子模块9/1(VC) -> Mux/10
  Demux/16 -> MMC子模块15/1(PWM)
  MMC子模块7/1(VC) -> Mux/8
  Demux/13 -> MMC子模块12/1(PWM)
  Demux/2 -> MMC子模块1/1(PWM)
  MMC子模块1/1(VC) -> Mux/2
  Demux/20 -> MMC子模块19/1(PWM)
  MMC子模块16/1(VC) -> Mux/17
  MMC子模块19/1(VC) -> Mux/20
  MMC子模块17/1(VC) -> Mux/18
  MMC子模块2/1(VC) -> Mux/3
  Demux/3 -> MMC子模块2/1(PWM)
  MMC子模块11/1(VC) -> Mux/12
  MMC子模块5/1(VC) -> Mux/6
  Demux/4 -> MMC子模块3/1(PWM)
  Demux/10 -> MMC子模块9/1(PWM)
  Demux/9 -> MMC子模块8/1(PWM)
  Demux/11 -> MMC子模块10/1(PWM)
  MMC子模块21/1(VC) -> Mux/22
  MMC子模块13/1(VC) -> Mux/14
  Demux/15 -> MMC子模块14/1(PWM)
  MMC子模块15/1(VC) -> Mux/16
  Demux/18 -> MMC子模块17/1(PWM)
  MMC子模块/1(VC) -> Mux/1
  MMC子模块12/1(VC) -> Mux/13
  Demux/12 -> MMC子模块11/1(PWM)
  Demux/6 -> MMC子模块5/1(PWM)
  Demux/8 -> MMC子模块7/1(PWM)
  Demux/7 -> MMC子模块6/1(PWM)
  MMC子模块10/1(VC) -> Mux/11
  MMC子模块8/1(VC) -> Mux/9
  MMC子模块3/1(VC) -> Mux/4
  PWM/1 -> Demux/1
  MMC子模块6/1(VC) -> Mux/7
  Demux/5 -> MMC子模块4/1(PWM)
  Demux/14 -> MMC子模块13/1(PWM)
  MMC子模块18/1(VC) -> Mux/19
  MMC子模块20/1(VC) -> Mux/21
  connections:
  MMC子模块6/LConn2 -- MMC子模块7/LConn1
  MMC子模块10/LConn1 -- MMC子模块9/LConn2
  MMC子模块2/LConn2 -- MMC子模块3/LConn1
  MMC子模块13/LConn2 -- MMC子模块14/LConn1
  MMC子模块5/LConn2 -- MMC子模块6/LConn1
  MMC子模块3/LConn2 -- MMC子模块4/LConn1
  MMC子模块10/LConn2 -- MMC子模块11/LConn1
  MMC子模块1/LConn2 -- MMC子模块2/LConn1
  MMC子模块7/LConn2 -- MMC子模块8/LConn1
  MMC子模块14/LConn2 -- MMC子模块15/LConn1
  MMC子模块19/LConn2 -- MMC子模块20/LConn1
  MMC子模块15/LConn2 -- MMC子模块16/LConn1
  MMC子模块20/LConn2 -- MMC子模块21/LConn1
  MMC子模块4/LConn2 -- MMC子模块5/LConn1
  MMC子模块12/LConn2 -- MMC子模块13/LConn1
  MMC子模块17/LConn2 -- MMC子模块18/LConn1
  MMC子模块11/LConn2 -- MMC子模块12/LConn1
  MMC子模块8/LConn2 -- MMC子模块9/LConn1
  MMC子模块/LConn2 -- MMC子模块1/LConn1
  MMC子模块18/LConn2 -- MMC子模块19/LConn1
  MMC子模块16/LConn2 -- MMC子模块17/LConn1
  V+/RConn1 -- MMC子模块/LConn1
  V-/RConn1 -- MMC子模块21/LConn2

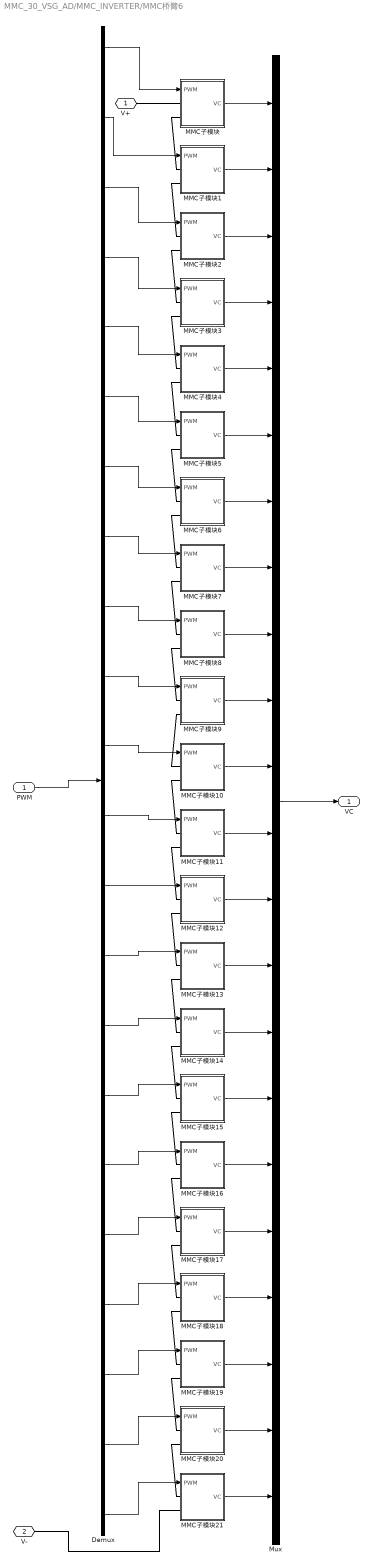
== system MMC_30_VSG_AD/MMC_INVERTER/MMC桥臂6 ==
  PWM : Inport
  Demux : Demux  Outputs=22
  MMC子模块 : Subsystem
  MMC子模块1 : Subsystem
  MMC子模块10 : Subsystem
  MMC子模块11 : Subsystem
  MMC子模块12 : Subsystem
  MMC子模块13 : Subsystem
  MMC子模块14 : Subsystem
  MMC子模块15 : Subsystem
  MMC子模块16 : Subsystem
  MMC子模块17 : Subsystem
  MMC子模块18 : Subsystem
  MMC子模块19 : Subsystem
  MMC子模块2 : Subsystem
  MMC子模块20 : Subsystem
  MMC子模块21 : Subsystem
  MMC子模块3 : Subsystem
  MMC子模块4 : Subsystem
  MMC子模块5 : Subsystem
  MMC子模块6 : Subsystem
  MMC子模块7 : Subsystem
  MMC子模块8 : Subsystem
  MMC子模块9 : Subsystem
  Mux : Mux  Inputs=22
  V+ : PMIOPort  Side=Left
  V- : PMIOPort  Port=2  Side=Left
  VC : Outport
  wires:
  MMC子模块20/1(VC) -> Mux/21
  MMC子模块18/1(VC) -> Mux/19
  Demux/14 -> MMC子模块13/1(PWM)
  Demux/5 -> MMC子模块4/1(PWM)
  MMC子模块6/1(VC) -> Mux/7
  PWM/1 -> Demux/1
  MMC子模块3/1(VC) -> Mux/4
  MMC子模块8/1(VC) -> Mux/9
  MMC子模块10/1(VC) -> Mux/11
  Demux/7 -> MMC子模块6/1(PWM)
  Demux/8 -> MMC子模块7/1(PWM)
  Demux/6 -> MMC子模块5/1(PWM)
  Demux/12 -> MMC子模块11/1(PWM)
  MMC子模块12/1(VC) -> Mux/13
  MMC子模块/1(VC) -> Mux/1
  Demux/18 -> MMC子模块17/1(PWM)
  MMC子模块15/1(VC) -> Mux/16
  Demux/15 -> MMC子模块14/1(PWM)
  MMC子模块13/1(VC) -> Mux/14
  MMC子模块21/1(VC) -> Mux/22
  Demux/11 -> MMC子模块10/1(PWM)
  Demux/9 -> MMC子模块8/1(PWM)
  Demux/10 -> MMC子模块9/1(PWM)
  Demux/4 -> MMC子模块3/1(PWM)
  MMC子模块5/1(VC) -> Mux/6
  MMC子模块11/1(VC) -> Mux/12
  Demux/3 -> MMC子模块2/1(PWM)
  MMC子模块2/1(VC) -> Mux/3
  MMC子模块17/1(VC) -> Mux/18
  MMC子模块19/1(VC) -> Mux/20
  MMC子模块16/1(VC) -> Mux/17
  Demux/20 -> MMC子模块19/1(PWM)
  MMC子模块1/1(VC) -> Mux/2
  Demux/2 -> MMC子模块1/1(PWM)
  Demux/13 -> MMC子模块12/1(PWM)
  MMC子模块7/1(VC) -> Mux/8
  Demux/16 -> MMC子模块15/1(PWM)
  MMC子模块9/1(VC) -> Mux/10
  Mux/1 -> VC/1
  MMC子模块14/1(VC) -> Mux/15
  Demux/1 -> MMC子模块/1(PWM)
  Demux/17 -> MMC子模块16/1(PWM)
  Demux/22 -> MMC子模块21/1(PWM)
  Demux/19 -> MMC子模块18/1(PWM)
  Demux/21 -> MMC子模块20/1(PWM)
  MMC子模块4/1(VC) -> Mux/5
  connections:
  V-/RConn1 -- MMC子模块21/LConn2
  V+/RConn1 -- MMC子模块/LConn1
  MMC子模块16/LConn2 -- MMC子模块17/LConn1
  MMC子模块18/LConn2 -- MMC子模块19/LConn1
  MMC子模块/LConn2 -- MMC子模块1/LConn1
  MMC子模块8/LConn2 -- MMC子模块9/LConn1
  MMC子模块11/LConn2 -- MMC子模块12/LConn1
  MMC子模块17/LConn2 -- MMC子模块18/LConn1
  MMC子模块12/LConn2 -- MMC子模块13/LConn1
  MMC子模块4/LConn2 -- MMC子模块5/LConn1
  MMC子模块20/LConn2 -- MMC子模块21/LConn1
  MMC子模块15/LConn2 -- MMC子模块16/LConn1
  MMC子模块19/LConn2 -- MMC子模块20/LConn1
  MMC子模块14/LConn2 -- MMC子模块15/LConn1
  MMC子模块7/LConn2 -- MMC子模块8/LConn1
  MMC子模块1/LConn2 -- MMC子模块2/LConn1
  MMC子模块10/LConn2 -- MMC子模块11/LConn1
  MMC子模块3/LConn2 -- MMC子模块4/LConn1
  MMC子模块5/LConn2 -- MMC子模块6/LConn1
  MMC子模块13/LConn2 -- MMC子模块14/LConn1
  MMC子模块2/LConn2 -- MMC子模块3/LConn1
  MMC子模块10/LConn1 -- MMC子模块9/LConn2
  MMC子模块6/LConn2 -- MMC子模块7/LConn1

== system MMC_30_VSG_AD/VSG控制/VSG无功控制-电压调节-调压 ==
  note: 线电压
  note: 相电压
  note: 6600线电压有效值
  note: Q*
  Un : Inport
  Vs : Inport  Port=2
  Qref : Inport  Port=3
  Qe : Inport  Port=4
  Constant2 : Constant  Value=5389
  Gain1 : Gain  Gain=0.02
  Gain2 : Gain  Gain=sqrt(3)
  Gain6 : Gain  Gain=2500
  Integrator : Integrator
  RMS : dspstat3/RMS  run=off  directionMode=Each column  dimension=1  InputProcessing=Columns as channels (frame based)  reset_popup=None
  Sum5 : Sum  Inputs=|+-
  Sum6 : Sum  Inputs=|++
  Sum7 : Sum  Inputs=|+-
  Sum8 : Sum  Inputs=|++
  E : Outport
  wires:
  Un/1 -> Sum5/1
  Vs/1 -> RMS/1
  RMS/1 -> Gain2/1
  Sum5/1 -> Gain6/1
  Gain6/1 -> Sum6/1
  Qref/1 -> Sum7/1
  Qe/1 -> Sum7/2
  Sum7/1 -> Sum6/2
  Sum6/1 -> Gain1/1
  Integrator/1 -> Sum8/1
  Constant2/1 -> Sum8/2
  Sum8/1 -> E/1
  Gain1/1 -> Integrator/1
  Gain2/1 -> Sum5/2

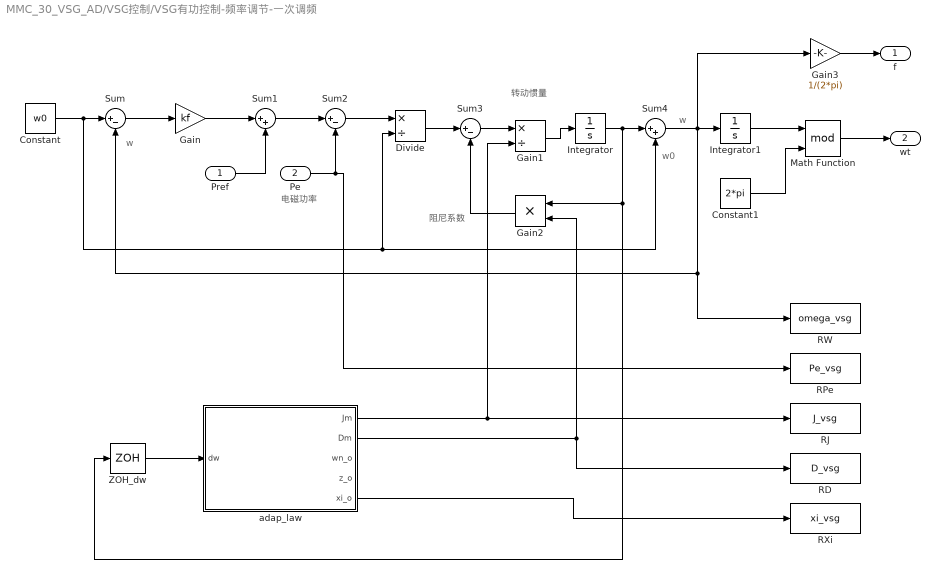
== system MMC_30_VSG_AD/VSG控制/VSG有功控制-频率调节-一次调频 ==
  note: w
  note: w0
  note: w
  note: 阻尼系数
  note: 转动惯量
  note: 电磁功率
  Pref : Inport
  Pe : Inport  Port=2
  Constant : Constant  Value=w0
  Constant1 : Constant  Value=2*pi
  Divide : Product  Inputs=*/
  Gain : Gain  Gain=kf
  Gain1 : Product  Inputs=*/
  Gain2 : Product
  Gain3 : Gain  Gain=1/(2*pi)
  Integrator : Integrator
  Integrator1 : Integrator  InitialCondition=delta0
  Math Function : Math  Operator=mod
  RD : ToWorkspace  VariableName=D_vsg  SaveFormat=Timeseries  SampleTime=Ts
  RJ : ToWorkspace  VariableName=J_vsg  SaveFormat=Timeseries  SampleTime=Ts
  RPe : ToWorkspace  VariableName=Pe_vsg  SaveFormat=Timeseries  SampleTime=Ts
  RW : ToWorkspace  VariableName=omega_vsg  SaveFormat=Timeseries  SampleTime=Ts
  RXi : ToWorkspace  VariableName=xi_vsg  SaveFormat=Timeseries  SampleTime=Ts
  Sum : Sum  Inputs=|+-
  Sum1 : Sum  Inputs=|++
  Sum2 : Sum  Inputs=|+-
  Sum3 : Sum  Inputs=|+-
  Sum4 : Sum  Inputs=|++
  ZOH_dw : ZeroOrderHold  SampleTime=Ts
  adap_law : MATLAB Function  TreatAsAtomicUnit=on
  f : Outport
  wt : Outport  Port=2
  wires:
  Sum/1 -> Gain/1
  Sum2/1 -> Divide/1
  Constant/1 -> Divide/2, Sum4/2, Sum/1
  Sum3/1 -> Gain1/1
  Pref/1 -> Sum1/2
  Pe/1 -> Sum2/2, RPe/1
  Integrator/1 -> ZOH_dw/1, Gain2/1, Sum4/1
  Math Function/1 -> wt/1
  Integrator1/1 -> Math Function/1
  Gain1/1 -> Integrator/1
  Constant1/1 -> Math Function/2
  Gain2/1 -> Sum3/2
  Sum4/1 -> RW/1, Sum/2, Gain3/1, Integrator1/1
  Sum1/1 -> Sum2/1
  Gain/1 -> Sum1/1
  Gain3/1 -> f/1
  Divide/1 -> Sum3/1
  ZOH_dw/1 -> adap_law/1(dw)
  adap_law/1(Jm) -> Gain1/2, RJ/1
  adap_law/2(Dm) -> Gain2/2, RD/1
  adap_law/5(xi_o) -> RXi/1

== system MMC_30_VSG_AD/环流抑制器/Subsystem1 ==
  In1 : Inport
  Gain1 : Gain  Gain=Kp
  Gain2 : Gain  Gain=Ki
  Integrator : Integrator
  Sum2 : Sum  Inputs=|+++
  Transfer Fcn : TransferFcn  Numerator=[2*Kr*wc 0]  Denominator=[1 2*wc wr^2]
  HL : Outport
  wires:
  Sum2/1 -> HL/1
  Gain1/1 -> Sum2/1
  In1/1 -> Transfer Fcn/1, Gain2/1, Gain1/1
  Transfer Fcn/1 -> Sum2/3
  Gain2/1 -> Integrator/1
  Integrator/1 -> Sum2/2

== system MMC_30_VSG_AD/环流抑制器/Subsystem2 ==
  In1 : Inport
  Gain1 : Gain  Gain=Kp
  Gain2 : Gain  Gain=Ki
  Integrator : Integrator
  Sum2 : Sum  Inputs=|+++
  Transfer Fcn : TransferFcn  Numerator=[2*Kr*wc 0]  Denominator=[1 2*wc wr^2]
  HL : Outport
  wires:
  Integrator/1 -> Sum2/2
  Gain2/1 -> Integrator/1
  Transfer Fcn/1 -> Sum2/3
  In1/1 -> Gain1/1, Gain2/1, Transfer Fcn/1
  Gain1/1 -> Sum2/1
  Sum2/1 -> HL/1

== system MMC_30_VSG_AD/环流抑制器/Subsystem3 ==
  In1 : Inport
  Gain1 : Gain  Gain=Kp
  Gain2 : Gain  Gain=Ki
  Integrator : Integrator
  Sum2 : Sum  Inputs=|+++
  Transfer Fcn : TransferFcn  Numerator=[2*Kr*wc 0]  Denominator=[1 2*wc wr^2]
  HL : Outport
  wires:
  Sum2/1 -> HL/1
  Gain1/1 -> Sum2/1
  In1/1 -> Transfer Fcn/1, Gain2/1, Gain1/1
  Transfer Fcn/1 -> Sum2/3
  Gain2/1 -> Integrator/1
  Integrator/1 -> Sum2/2
